simulink model "ADCS_FSM_v1_test"  (R2025b)
settings: Solver=VariableStepAuto  StartTime=0.0  StopTime=t0  FixedStep=0.1  MaxStep=0.1  RelTol=1e-3
model workspace (MAT data in the model file):
  i = 8
  omega_thr = 1
  simIn = Simulink.SimulationInput
  simIn.ExternalInput = Simulink.SimulationData.Dataset
  simIn.ExternalInput.any.Name = ''
  simIn.ExternalInput.any.Version = 3
  simIn.ExternalInput.any.Storage = Simulink.SimulationData.Storage.RamDatasetStorage
  simIn.ExternalInput.any.Storage.any.Version = 2
  simIn.ExternalInput.any.Storage.any.Elements{1} = timeseries
  simIn.ExternalInput.any.Storage.any.Elements{1}.Name = 'u1'
  simIn.ExternalInput.any.Storage.any.Elements{1}.DataInfo = tsdata.datametadata
  simIn.ExternalInput.any.Storage.any.Elements{1}.DataInfo.Interpolation = tsdata.interpolation
  simIn.ExternalInput.any.Storage.any.Elements{1}.DataInfo.Interpolation.Fhandle : function handle (value not decoded)
  simIn.ExternalInput.any.Storage.any.Elements{1}.DataInfo.Interpolation.Name = 'linear'
  simIn.ExternalInput.any.Storage.any.Elements{1}.TimeInfo = tsdata.timemetadata
  simIn.ExternalInput.any.Storage.any.Elements{1}.TimeInfo.Length = 101
  simIn.ExternalInput.any.Storage.any.Elements{1}.TimeInfo.DuplicateTimes = 0
  simIn.ExternalInput.any.Storage.any.Elements{1}.TimeInfo.Time_ = [0; 0.1; 0.2; 0.3; 0.4; 0.5; 0.6; 0.7; 0.8; 0.9; 1; 1.1; 1.2; 1.3; 1.4; 1.5; 1.6; 1.7; 1.8; 1.9; 2; 2.1; 2.2; 2.3; 2.4; 2.5; 2.6; 2.7; 2.8; 2.9; 3; 3.1; 3.2; 3.3; 3.4; 3.5; 3.6; 3.7; 3.8; 3.9; 4; 4.1; 4.2; 4.3; 4.4; 4.5; 4.6; 4.7; 4.8; 4.9; 5; 5.1; 5.2; 5.3; 5.4; 5.5; 5.6; 5.7; 5.8; 5.9; 6; 6.1; 6.2; 6.3; 6.4; 6.5; 6.6; 6.7; 6.8; 6.9; 7; 7.1; 7.2; 7.3; 7.4; 7.5; 7.6; 7.7; 7.8; 7.9; 8; 8.1; 8.2; 8.3; 8.4; 8.5; 8.6; 8.7; 8.8; 8.9; 9; 9.1; 9.2; 9.3; 9.4; 9.5; 9.6; 9.7; 9.8; 9.9; 10]
  simIn.ExternalInput.any.Storage.any.Elements{1}.TimeInfo.Initialized = 1
  simIn.ExternalInput.any.Storage.any.Elements{1}.QualityInfo = tsdata.qualmetadata
  simIn.ExternalInput.any.Storage.any.Elements{1}.Data_ = [12; 12; 12; 12; 12; 12; 12; 12; 12; 12; 12; 12; 12; 12; 12; 12; 12; 12; 12; 12; 12; 12; 12; 12; 12; 12; 12; 12; 12; 12; 12; 12; 12; 12; 12; 12; 12; 12; 12; 12; 12; 12; 12; 12; 12; 12; 12; 12; 12; 12; 12; 12; 12; 12; 12; 12; 12; 12; 12; 12; 12; 12; 12; 12; 12; 12; 12; 12; 12; 12; 12; 12; 12; 12; 12; 12; 12; 12; 12; 12; 12; 12; 12; 12; 12; 12; 12; 12; 12; 12; 12; 12; 12; 12; 12; 12; 12; 12; 12; 12; 12]
  simIn.ExternalInput.any.Storage.any.Elements{2} = timeseries
  simIn.ExternalInput.any.Storage.any.Elements{2}.Name = 'u2'
  simIn.ExternalInput.any.Storage.any.Elements{2}.DataInfo = tsdata.datametadata
  simIn.ExternalInput.any.Storage.any.Elements{2}.DataInfo.Interpolation = tsdata.interpolation
  simIn.ExternalInput.any.Storage.any.Elements{2}.DataInfo.Interpolation.Fhandle : function handle (value not decoded)
  simIn.ExternalInput.any.Storage.any.Elements{2}.DataInfo.Interpolation.Name = 'linear'
  simIn.ExternalInput.any.Storage.any.Elements{2}.TimeInfo = tsdata.timemetadata
  simIn.ExternalInput.any.Storage.any.Elements{2}.TimeInfo.Length = 101
  simIn.ExternalInput.any.Storage.any.Elements{2}.TimeInfo.DuplicateTimes = 0
  simIn.ExternalInput.any.Storage.any.Elements{2}.TimeInfo.Time_ = [0; 0.1; 0.2; 0.3; 0.4; 0.5; 0.6; 0.7; 0.8; 0.9; 1; 1.1; 1.2; 1.3; 1.4; 1.5; 1.6; 1.7; 1.8; 1.9; 2; 2.1; 2.2; 2.3; 2.4; 2.5; 2.6; 2.7; 2.8; 2.9; 3; 3.1; 3.2; 3.3; 3.4; 3.5; 3.6; 3.7; 3.8; 3.9; 4; 4.1; 4.2; 4.3; 4.4; 4.5; 4.6; 4.7; 4.8; 4.9; 5; 5.1; 5.2; 5.3; 5.4; 5.5; 5.6; 5.7; 5.8; 5.9; 6; 6.1; 6.2; 6.3; 6.4; 6.5; 6.6; 6.7; 6.8; 6.9; 7; 7.1; 7.2; 7.3; 7.4; 7.5; 7.6; 7.7; 7.8; 7.9; 8; 8.1; 8.2; 8.3; 8.4; 8.5; 8.6; 8.7; 8.8; 8.9; 9; 9.1; 9.2; 9.3; 9.4; 9.5; 9.6; 9.7; 9.8; 9.9; 10]
  simIn.ExternalInput.any.Storage.any.Elements{2}.TimeInfo.Initialized = 1
  simIn.ExternalInput.any.Storage.any.Elements{2}.QualityInfo = tsdata.qualmetadata
  simIn.ExternalInput.any.Storage.any.Elements{2}.Data_ = [1; 1; 1; 1; 1; 1; 1; 1; 1; 1; 1; 1; 1; 1; 1; 1; 1; 1; 1; 1; 1; 1; 1; 1; 1; 1; 1; 1; 1; 1; 1; 1; 1; 1; 1; 1; 1; 1; 1; 1; 1; 1; 1; 1; 1; 1; 1; 1; 1; 1; 1; 1; 1; 1; 1; 1; 1; 1; 1; 1; 1; 1; 1; 1; 1; 1; 1; 1; 1; 1; 1; 1; 1; 1; 1; 1; 1; 1; 1; 1; 1; 1; 1; 1; 1; 1; 1; 1; 1; 1; 1; 1; 1; 1; 1; 1; 1; 1; 1; 1; 1]
  simIn.ExternalInput.any.Storage.any.Elements{3} = timeseries
  simIn.ExternalInput.any.Storage.any.Elements{3}.Name = 'u3'
  simIn.ExternalInput.any.Storage.any.Elements{3}.DataInfo = tsdata.datametadata
  simIn.ExternalInput.any.Storage.any.Elements{3}.DataInfo.Interpolation = tsdata.interpolation
  simIn.ExternalInput.any.Storage.any.Elements{3}.DataInfo.Interpolation.Fhandle : function handle (value not decoded)
  simIn.ExternalInput.any.Storage.any.Elements{3}.DataInfo.Interpolation.Name = 'linear'
  simIn.ExternalInput.any.Storage.any.Elements{3}.TimeInfo = tsdata.timemetadata
  simIn.ExternalInput.any.Storage.any.Elements{3}.TimeInfo.Length = 101
  simIn.ExternalInput.any.Storage.any.Elements{3}.TimeInfo.DuplicateTimes = 0
  simIn.ExternalInput.any.Storage.any.Elements{3}.TimeInfo.Time_ = [0; 0.1; 0.2; 0.3; 0.4; 0.5; 0.6; 0.7; 0.8; 0.9; 1; 1.1; 1.2; 1.3; 1.4; 1.5; 1.6; 1.7; 1.8; 1.9; 2; 2.1; 2.2; 2.3; 2.4; 2.5; 2.6; 2.7; 2.8; 2.9; 3; 3.1; 3.2; 3.3; 3.4; 3.5; 3.6; 3.7; 3.8; 3.9; 4; 4.1; 4.2; 4.3; 4.4; 4.5; 4.6; 4.7; 4.8; 4.9; 5; 5.1; 5.2; 5.3; 5.4; 5.5; 5.6; 5.7; 5.8; 5.9; 6; 6.1; 6.2; 6.3; 6.4; 6.5; 6.6; 6.7; 6.8; 6.9; 7; 7.1; 7.2; 7.3; 7.4; 7.5; 7.6; 7.7; 7.8; 7.9; 8; 8.1; 8.2; 8.3; 8.4; 8.5; 8.6; 8.7; 8.8; 8.9; 9; 9.1; 9.2; 9.3; 9.4; 9.5; 9.6; 9.7; 9.8; 9.9; 10]
  simIn.ExternalInput.any.Storage.any.Elements{3}.TimeInfo.Initialized = 1
  simIn.ExternalInput.any.Storage.any.Elements{3}.QualityInfo = tsdata.qualmetadata
  simIn.ExternalInput.any.Storage.any.Elements{3}.Data_ = [0; 0; 0; 0; 0; 0; 0; 0; 0; 0; 0; 0; 0; 0; 0; 0; 0; 0; 0; 0; 0; 0; 0; 0; 0; 0; 0; 0; 0; 0; 0; 0; 0; 0; 0; 0; 0; 0; 0; 0; 0; 0; 0; 0; 0; 0; 0; 0; 0; 0; 0; 0; 0; 0; 0; 0; 0; 0; 0; 0; 0; 0; 0; 0; 0; 0; 0; 0; 0; 0; 0; 0; 0; 0; 0; 0; 0; 0; 0; 0; 0; 0; 0; 0; 0; 0; 0; 0; 0; 0; 0; 0; 0; 0; 0; 0; 0; 0; 0; 0; 0]
  simIn.ExternalInput.any.Storage.any.Elements{4} = timeseries
  simIn.ExternalInput.any.Storage.any.Elements{4}.Name = 'u4'
  simIn.ExternalInput.any.Storage.any.Elements{4}.DataInfo = tsdata.datametadata
  simIn.ExternalInput.any.Storage.any.Elements{4}.DataInfo.Interpolation = tsdata.interpolation
  simIn.ExternalInput.any.Storage.any.Elements{4}.DataInfo.Interpolation.Fhandle : function handle (value not decoded)
  simIn.ExternalInput.any.Storage.any.Elements{4}.DataInfo.Interpolation.Name = 'linear'
  simIn.ExternalInput.any.Storage.any.Elements{4}.TimeInfo = tsdata.timemetadata
  simIn.ExternalInput.any.Storage.any.Elements{4}.TimeInfo.Length = 101
  simIn.ExternalInput.any.Storage.any.Elements{4}.TimeInfo.DuplicateTimes = 0
  simIn.ExternalInput.any.Storage.any.Elements{4}.TimeInfo.Time_ = [0; 0.1; 0.2; 0.3; 0.4; 0.5; 0.6; 0.7; 0.8; 0.9; 1; 1.1; 1.2; 1.3; 1.4; 1.5; 1.6; 1.7; 1.8; 1.9; 2; 2.1; 2.2; 2.3; 2.4; 2.5; 2.6; 2.7; 2.8; 2.9; 3; 3.1; 3.2; 3.3; 3.4; 3.5; 3.6; 3.7; 3.8; 3.9; 4; 4.1; 4.2; 4.3; 4.4; 4.5; 4.6; 4.7; 4.8; 4.9; 5; 5.1; 5.2; 5.3; 5.4; 5.5; 5.6; 5.7; 5.8; 5.9; 6; 6.1; 6.2; 6.3; 6.4; 6.5; 6.6; 6.7; 6.8; 6.9; 7; 7.1; 7.2; 7.3; 7.4; 7.5; 7.6; 7.7; 7.8; 7.9; 8; 8.1; 8.2; 8.3; 8.4; 8.5; 8.6; 8.7; 8.8; 8.9; 9; 9.1; 9.2; 9.3; 9.4; 9.5; 9.6; 9.7; 9.8; 9.9; 10]
  simIn.ExternalInput.any.Storage.any.Elements{4}.TimeInfo.Initialized = 1
  simIn.ExternalInput.any.Storage.any.Elements{4}.QualityInfo = tsdata.qualmetadata
  simIn.ExternalInput.any.Storage.any.Elements{4}.Data_ = [1; 1; 1; 1; 1; 1; 1; 1; 1; 1; 1; 1; 1; 1; 1; 1; 1; 1; 1; 1; 1; 1; 1; 1; 1; 1; 1; 1; 1; 1; 1; 1; 1; 1; 1; 1; 1; 1; 1; 1; 1; 1; 1; 1; 1; 1; 1; 1; 1; 1; 1; 1; 1; 1; 1; 1; 1; 1; 1; 1; 1; 1; 1; 1; 1; 1; 1; 1; 1; 1; 1; 1; 1; 1; 1; 1; 1; 1; 1; 1; 1; 1; 1; 1; 1; 1; 1; 1; 1; 1; 1; 1; 1; 1; 1; 1; 1; 1; 1; 1; 1]
  simIn.ExternalInput.any.Storage.any.Elements{5} = timeseries
  simIn.ExternalInput.any.Storage.any.Elements{5}.Name = 'u5'
  simIn.ExternalInput.any.Storage.any.Elements{5}.DataInfo = tsdata.datametadata
  simIn.ExternalInput.any.Storage.any.Elements{5}.DataInfo.Interpolation = tsdata.interpolation
  simIn.ExternalInput.any.Storage.any.Elements{5}.DataInfo.Interpolation.Fhandle : function handle (value not decoded)
  simIn.ExternalInput.any.Storage.any.Elements{5}.DataInfo.Interpolation.Name = 'linear'
  simIn.ExternalInput.any.Storage.any.Elements{5}.TimeInfo = tsdata.timemetadata
  simIn.ExternalInput.any.Storage.any.Elements{5}.TimeInfo.Length = 101
  simIn.ExternalInput.any.Storage.any.Elements{5}.TimeInfo.DuplicateTimes = 0
  simIn.ExternalInput.any.Storage.any.Elements{5}.TimeInfo.Time_ = [0; 0.1; 0.2; 0.3; 0.4; 0.5; 0.6; 0.7; 0.8; 0.9; 1; 1.1; 1.2; 1.3; 1.4; 1.5; 1.6; 1.7; 1.8; 1.9; 2; 2.1; 2.2; 2.3; 2.4; 2.5; 2.6; 2.7; 2.8; 2.9; 3; 3.1; 3.2; 3.3; 3.4; 3.5; 3.6; 3.7; 3.8; 3.9; 4; 4.1; 4.2; 4.3; 4.4; 4.5; 4.6; 4.7; 4.8; 4.9; 5; 5.1; 5.2; 5.3; 5.4; 5.5; 5.6; 5.7; 5.8; 5.9; 6; 6.1; 6.2; 6.3; 6.4; 6.5; 6.6; 6.7; 6.8; 6.9; 7; 7.1; 7.2; 7.3; 7.4; 7.5; 7.6; 7.7; 7.8; 7.9; 8; 8.1; 8.2; 8.3; 8.4; 8.5; 8.6; 8.7; 8.8; 8.9; 9; 9.1; 9.2; 9.3; 9.4; 9.5; 9.6; 9.7; 9.8; 9.9; 10]
  simIn.ExternalInput.any.Storage.any.Elements{5}.TimeInfo.Initialized = 1
  simIn.ExternalInput.any.Storage.any.Elements{5}.QualityInfo = tsdata.qualmetadata
  simIn.ExternalInput.any.Storage.any.Elements{5}.Data_ = [0; 0; 0; 0; 0; 0; 0; 0; 0; 0; 0; 0; 0; 0; 0; 0; 0; 0; 0; 0; 0; 0; 0; 0; 0; 0; 0; 0; 0; 0; 0; 0; 0; 0; 0; 0; 0; 0; 0; 0; 0; 0; 0; 0; 0; 0; 0; 0; 0; 0; 0; 0; 0; 0; 0; 0; 0; 0; 0; 0; 0; 0; 0; 0; 0; 0; 0; 0; 0; 0; 0; 0; 0; 0; 0; 0; 0; 0; 0; 0; 0; 0; 0; 0; 0; 0; 0; 0; 0; 0; 0; 0; 0; 0; 0; 0; 0; 0; 0; 0; 0]
  simIn.ExternalInput.any.Storage.any.Elements{6} = timeseries
  simIn.ExternalInput.any.Storage.any.Elements{6}.Name = 'u6'
  simIn.ExternalInput.any.Storage.any.Elements{6}.DataInfo = tsdata.datametadata
  simIn.ExternalInput.any.Storage.any.Elements{6}.DataInfo.Interpolation = tsdata.interpolation
  simIn.ExternalInput.any.Storage.any.Elements{6}.DataInfo.Interpolation.Fhandle : function handle (value not decoded)
  simIn.ExternalInput.any.Storage.any.Elements{6}.DataInfo.Interpolation.Name = 'linear'
  simIn.ExternalInput.any.Storage.any.Elements{6}.TimeInfo = tsdata.timemetadata
  simIn.ExternalInput.any.Storage.any.Elements{6}.TimeInfo.Length = 101
  simIn.ExternalInput.any.Storage.any.Elements{6}.TimeInfo.DuplicateTimes = 0
  simIn.ExternalInput.any.Storage.any.Elements{6}.TimeInfo.Time_ = [0; 0.1; 0.2; 0.3; 0.4; 0.5; 0.6; 0.7; 0.8; 0.9; 1; 1.1; 1.2; 1.3; 1.4; 1.5; 1.6; 1.7; 1.8; 1.9; 2; 2.1; 2.2; 2.3; 2.4; 2.5; 2.6; 2.7; 2.8; 2.9; 3; 3.1; 3.2; 3.3; 3.4; 3.5; 3.6; 3.7; 3.8; 3.9; 4; 4.1; 4.2; 4.3; 4.4; 4.5; 4.6; 4.7; 4.8; 4.9; 5; 5.1; 5.2; 5.3; 5.4; 5.5; 5.6; 5.7; 5.8; 5.9; 6; 6.1; 6.2; 6.3; 6.4; 6.5; 6.6; 6.7; 6.8; 6.9; 7; 7.1; 7.2; 7.3; 7.4; 7.5; 7.6; 7.7; 7.8; 7.9; 8; 8.1; 8.2; 8.3; 8.4; 8.5; 8.6; 8.7; 8.8; 8.9; 9; 9.1; 9.2; 9.3; 9.4; 9.5; 9.6; 9.7; 9.8; 9.9; 10]
  simIn.ExternalInput.any.Storage.any.Elements{6}.TimeInfo.Initialized = 1
  simIn.ExternalInput.any.Storage.any.Elements{6}.QualityInfo = tsdata.qualmetadata
  simIn.ExternalInput.any.Storage.any.Elements{6}.Data_ = [1; 1; 1; 1; 1; 1; 1; 1; 1; 1; 1; 1; 1; 1; 1; 1; 1; 1; 1; 1; 1; 1; 1; 1; 1; 1; 1; 1; 1; 1; 1; 1; 1; 1; 1; 1; 1; 1; 1; 1; 1; 1; 1; 1; 1; 1; 1; 1; 1; 1; 1; 1; 1; 1; 1; 1; 1; 1; 1; 1; 1; 1; 1; 1; 1; 1; 1; 1; 1; 1; 1; 1; 1; 1; 1; 1; 1; 1; 1; 1; 1; 1; 1; 1; 1; 1; 1; 1; 1; 1; 1; 1; 1; 1; 1; 1; 1; 1; 1; 1; 1]
  simIn.ExternalInput.any.Storage.any.Elements{7} = timeseries
  simIn.ExternalInput.any.Storage.any.Elements{7}.Name = 'u7'
  simIn.ExternalInput.any.Storage.any.Elements{7}.DataInfo = tsdata.datametadata
  simIn.ExternalInput.any.Storage.any.Elements{7}.DataInfo.Interpolation = tsdata.interpolation
  simIn.ExternalInput.any.Storage.any.Elements{7}.DataInfo.Interpolation.Fhandle : function handle (value not decoded)
  simIn.ExternalInput.any.Storage.any.Elements{7}.DataInfo.Interpolation.Name = 'linear'
  simIn.ExternalInput.any.Storage.any.Elements{7}.TimeInfo = tsdata.timemetadata
  simIn.ExternalInput.any.Storage.any.Elements{7}.TimeInfo.Length = 101
  simIn.ExternalInput.any.Storage.any.Elements{7}.TimeInfo.DuplicateTimes = 0
  simIn.ExternalInput.any.Storage.any.Elements{7}.TimeInfo.Time_ = [0; 0.1; 0.2; 0.3; 0.4; 0.5; 0.6; 0.7; 0.8; 0.9; 1; 1.1; 1.2; 1.3; 1.4; 1.5; 1.6; 1.7; 1.8; 1.9; 2; 2.1; 2.2; 2.3; 2.4; 2.5; 2.6; 2.7; 2.8; 2.9; 3; 3.1; 3.2; 3.3; 3.4; 3.5; 3.6; 3.7; 3.8; 3.9; 4; 4.1; 4.2; 4.3; 4.4; 4.5; 4.6; 4.7; 4.8; 4.9; 5; 5.1; 5.2; 5.3; 5.4; 5.5; 5.6; 5.7; 5.8; 5.9; 6; 6.1; 6.2; 6.3; 6.4; 6.5; 6.6; 6.7; 6.8; 6.9; 7; 7.1; 7.2; 7.3; 7.4; 7.5; 7.6; 7.7; 7.8; 7.9; 8; 8.1; 8.2; 8.3; 8.4; 8.5; 8.6; 8.7; 8.8; 8.9; 9; 9.1; 9.2; 9.3; 9.4; 9.5; 9.6; 9.7; 9.8; 9.9; 10]
  simIn.ExternalInput.any.Storage.any.Elements{7}.TimeInfo.Initialized = 1
  simIn.ExternalInput.any.Storage.any.Elements{7}.QualityInfo = tsdata.qualmetadata
  simIn.ExternalInput.any.Storage.any.Elements{7}.Data_ = [1; 1; 1; 1; 1; 1; 1; 1; 1; 1; 1; 1; 1; 1; 1; 1; 1; 1; 1; 1; 1; 1; 1; 1; 1; 1; 1; 1; 1; 1; 1; 1; 1; 1; 1; 1; 1; 1; 1; 1; 1; 1; 1; 1; 1; 1; 1; 1; 1; 1; 1; 1; 1; 1; 1; 1; 1; 1; 1; 1; 1; 1; 1; 1; 1; 1; 1; 1; 1; 1; 1; 1; 1; 1; 1; 1; 1; 1; 1; 1; 1; 1; 1; 1; 1; 1; 1; 1; 1; 1; 1; 1; 1; 1; 1; 1; 1; 1; 1; 1; 1]
  simIn.ExternalInput.any.Storage.any.Elements{8} = timeseries
  simIn.ExternalInput.any.Storage.any.Elements{8}.Name = 'u8'
  simIn.ExternalInput.any.Storage.any.Elements{8}.DataInfo = tsdata.datametadata
  simIn.ExternalInput.any.Storage.any.Elements{8}.DataInfo.Interpolation = tsdata.interpolation
  simIn.ExternalInput.any.Storage.any.Elements{8}.DataInfo.Interpolation.Fhandle : function handle (value not decoded)
  simIn.ExternalInput.any.Storage.any.Elements{8}.DataInfo.Interpolation.Name = 'linear'
  simIn.ExternalInput.any.Storage.any.Elements{8}.TimeInfo = tsdata.timemetadata
  simIn.ExternalInput.any.Storage.any.Elements{8}.TimeInfo.Length = 101
  simIn.ExternalInput.any.Storage.any.Elements{8}.TimeInfo.DuplicateTimes = 0
  simIn.ExternalInput.any.Storage.any.Elements{8}.TimeInfo.Time_ = [0; 0.1; 0.2; 0.3; 0.4; 0.5; 0.6; 0.7; 0.8; 0.9; 1; 1.1; 1.2; 1.3; 1.4; 1.5; 1.6; 1.7; 1.8; 1.9; 2; 2.1; 2.2; 2.3; 2.4; 2.5; 2.6; 2.7; 2.8; 2.9; 3; 3.1; 3.2; 3.3; 3.4; 3.5; 3.6; 3.7; 3.8; 3.9; 4; 4.1; 4.2; 4.3; 4.4; 4.5; 4.6; 4.7; 4.8; 4.9; 5; 5.1; 5.2; 5.3; 5.4; 5.5; 5.6; 5.7; 5.8; 5.9; 6; 6.1; 6.2; 6.3; 6.4; 6.5; 6.6; 6.7; 6.8; 6.9; 7; 7.1; 7.2; 7.3; 7.4; 7.5; 7.6; 7.7; 7.8; 7.9; 8; 8.1; 8.2; 8.3; 8.4; 8.5; 8.6; 8.7; 8.8; 8.9; 9; 9.1; 9.2; 9.3; 9.4; 9.5; 9.6; 9.7; 9.8; 9.9; 10]
  simIn.ExternalInput.any.Storage.any.Elements{8}.TimeInfo.Initialized = 1
  simIn.ExternalInput.any.Storage.any.Elements{8}.QualityInfo = tsdata.qualmetadata
  simIn.ExternalInput.any.Storage.any.Elements{8}.Data_ = [0; 0; 0; 0; 0; 0; 0; 0; 0; 0; 0; 0; 0; 0; 0; 0; 0; 0; 0; 0; 0; 0; 0; 0; 0; 0; 0; 0; 0; 0; 0; 0; 0; 0; 0; 0; 0; 0; 0; 0; 0; 0; 0; 0; 0; 0; 0; 0; 0; 0; 0; 0; 0; 0; 0; 0; 0; 0; 0; 0; 0; 0; 0; 0; 0; 0; 0; 0; 0; 0; 0; 0; 0; 0; 0; 0; 0; 0; 0; 0; 0; 0; 0; 0; 0; 0; 0; 0; 0; 0; 0; 0; 0; 0; 0; 0; 0; 0; 0; 0; 0]
  simIn.ExternalInput.any.Storage.any.Elements{9} = timeseries
  simIn.ExternalInput.any.Storage.any.Elements{9}.Name = 'u9'
  simIn.ExternalInput.any.Storage.any.Elements{9}.DataInfo = tsdata.datametadata
  simIn.ExternalInput.any.Storage.any.Elements{9}.DataInfo.Interpolation = tsdata.interpolation
  simIn.ExternalInput.any.Storage.any.Elements{9}.DataInfo.Interpolation.Fhandle : function handle (value not decoded)
  simIn.ExternalInput.any.Storage.any.Elements{9}.DataInfo.Interpolation.Name = 'linear'
  simIn.ExternalInput.any.Storage.any.Elements{9}.TimeInfo = tsdata.timemetadata
  simIn.ExternalInput.any.Storage.any.Elements{9}.TimeInfo.Length = 101
  simIn.ExternalInput.any.Storage.any.Elements{9}.TimeInfo.DuplicateTimes = 0
  simIn.ExternalInput.any.Storage.any.Elements{9}.TimeInfo.Time_ = [0; 0.1; 0.2; 0.3; 0.4; 0.5; 0.6; 0.7; 0.8; 0.9; 1; 1.1; 1.2; 1.3; 1.4; 1.5; 1.6; 1.7; 1.8; 1.9; 2; 2.1; 2.2; 2.3; 2.4; 2.5; 2.6; 2.7; 2.8; 2.9; 3; 3.1; 3.2; 3.3; 3.4; 3.5; 3.6; 3.7; 3.8; 3.9; 4; 4.1; 4.2; 4.3; 4.4; 4.5; 4.6; 4.7; 4.8; 4.9; 5; 5.1; 5.2; 5.3; 5.4; 5.5; 5.6; 5.7; 5.8; 5.9; 6; 6.1; 6.2; 6.3; 6.4; 6.5; 6.6; 6.7; 6.8; 6.9; 7; 7.1; 7.2; 7.3; 7.4; 7.5; 7.6; 7.7; 7.8; 7.9; 8; 8.1; 8.2; 8.3; 8.4; 8.5; 8.6; 8.7; 8.8; 8.9; 9; 9.1; 9.2; 9.3; 9.4; 9.5; 9.6; 9.7; 9.8; 9.9; 10]
  simIn.ExternalInput.any.Storage.any.Elements{9}.TimeInfo.Initialized = 1
  simIn.ExternalInput.any.Storage.any.Elements{9}.QualityInfo = tsdata.qualmetadata
  simIn.ExternalInput.any.Storage.any.Elements{9}.Data_ = [1; 1; 1; 1; 1; 1; 1; 1; 1; 1; 1; 1; 1; 1; 1; 1; 1; 1; 1; 1; 1; 1; 1; 1; 1; 1; 1; 1; 1; 1; 1; 1; 1; 1; 1; 1; 1; 1; 1; 1; 1; 1; 1; 1; 1; 1; 1; 1; 1; 1; 1; 1; 1; 1; 1; 1; 1; 1; 1; 1; 1; 1; 1; 1; 1; 1; 1; 1; 1; 1; 1; 1; 1; 1; 1; 1; 1; 1; 1; 1; 1; 1; 1; 1; 1; 1; 1; 1; 1; 1; 1; 1; 1; 1; 1; 1; 1; 1; 1; 1; 1]
  simIn.ExternalInput.any.Storage.any.Elements{10} = timeseries
  simIn.ExternalInput.any.Storage.any.Elements{10}.Name = 'u10'
  simIn.ExternalInput.any.Storage.any.Elements{10}.DataInfo = tsdata.datametadata
  simIn.ExternalInput.any.Storage.any.Elements{10}.DataInfo.Interpolation = tsdata.interpolation
  simIn.ExternalInput.any.Storage.any.Elements{10}.DataInfo.Interpolation.Fhandle : function handle (value not decoded)
  simIn.ExternalInput.any.Storage.any.Elements{10}.DataInfo.Interpolation.Name = 'linear'
  simIn.ExternalInput.any.Storage.any.Elements{10}.TimeInfo = tsdata.timemetadata
  simIn.ExternalInput.any.Storage.any.Elements{10}.TimeInfo.Length = 101
  simIn.ExternalInput.any.Storage.any.Elements{10}.TimeInfo.DuplicateTimes = 0
  simIn.ExternalInput.any.Storage.any.Elements{10}.TimeInfo.Time_ = [0; 0.1; 0.2; 0.3; 0.4; 0.5; 0.6; 0.7; 0.8; 0.9; 1; 1.1; 1.2; 1.3; 1.4; 1.5; 1.6; 1.7; 1.8; 1.9; 2; 2.1; 2.2; 2.3; 2.4; 2.5; 2.6; 2.7; 2.8; 2.9; 3; 3.1; 3.2; 3.3; 3.4; 3.5; 3.6; 3.7; 3.8; 3.9; 4; 4.1; 4.2; 4.3; 4.4; 4.5; 4.6; 4.7; 4.8; 4.9; 5; 5.1; 5.2; 5.3; 5.4; 5.5; 5.6; 5.7; 5.8; 5.9; 6; 6.1; 6.2; 6.3; 6.4; 6.5; 6.6; 6.7; 6.8; 6.9; 7; 7.1; 7.2; 7.3; 7.4; 7.5; 7.6; 7.7; 7.8; 7.9; 8; 8.1; 8.2; 8.3; 8.4; 8.5; 8.6; 8.7; 8.8; 8.9; 9; 9.1; 9.2; 9.3; 9.4; 9.5; 9.6; 9.7; 9.8; 9.9; 10]
  simIn.ExternalInput.any.Storage.any.Elements{10}.TimeInfo.Initialized = 1
  simIn.ExternalInput.any.Storage.any.Elements{10}.QualityInfo = tsdata.qualmetadata
  simIn.ExternalInput.any.Storage.any.Elements{10}.Data_ = [0; 0; 0; 0; 0; 0; 0; 0; 0; 0; 0; 0; 0; 0; 0; 0; 0; 0; 0; 0; 0; 0; 0; 0; 0; 0; 0; 0; 0; 0; 0; 0; 0; 0; 0; 0; 0; 0; 0; 0; 0; 0; 0; 0; 0; 0; 0; 0; 0; 0; 0; 0; 0; 0; 0; 0; 0; 0; 0; 0; 0; 0; 0; 0; 0; 0; 0; 0; 0; 0; 0; 0; 0; 0; 0; 0; 0; 0; 0; 0; 0; 0; 0; 0; 0; 0; 0; 0; 0; 0; 0; 0; 0; 0; 0; 0; 0; 0; 0; 0; 0]
  simIn.ExternalInput.any.Storage.any.Elements{11} = timeseries
  simIn.ExternalInput.any.Storage.any.Elements{11}.Name = 'u11'
  simIn.ExternalInput.any.Storage.any.Elements{11}.DataInfo = tsdata.datametadata
  simIn.ExternalInput.any.Storage.any.Elements{11}.DataInfo.Interpolation = tsdata.interpolation
  simIn.ExternalInput.any.Storage.any.Elements{11}.DataInfo.Interpolation.Fhandle : function handle (value not decoded)
  simIn.ExternalInput.any.Storage.any.Elements{11}.DataInfo.Interpolation.Name = 'linear'
  simIn.ExternalInput.any.Storage.any.Elements{11}.TimeInfo = tsdata.timemetadata
  simIn.ExternalInput.any.Storage.any.Elements{11}.TimeInfo.Length = 101
  simIn.ExternalInput.any.Storage.any.Elements{11}.TimeInfo.DuplicateTimes = 0
  simIn.ExternalInput.any.Storage.any.Elements{11}.TimeInfo.Time_ = [0; 0.1; 0.2; 0.3; 0.4; 0.5; 0.6; 0.7; 0.8; 0.9; 1; 1.1; 1.2; 1.3; 1.4; 1.5; 1.6; 1.7; 1.8; 1.9; 2; 2.1; 2.2; 2.3; 2.4; 2.5; 2.6; 2.7; 2.8; 2.9; 3; 3.1; 3.2; 3.3; 3.4; 3.5; 3.6; 3.7; 3.8; 3.9; 4; 4.1; 4.2; 4.3; 4.4; 4.5; 4.6; 4.7; 4.8; 4.9; 5; 5.1; 5.2; 5.3; 5.4; 5.5; 5.6; 5.7; 5.8; 5.9; 6; 6.1; 6.2; 6.3; 6.4; 6.5; 6.6; 6.7; 6.8; 6.9; 7; 7.1; 7.2; 7.3; 7.4; 7.5; 7.6; 7.7; 7.8; 7.9; 8; 8.1; 8.2; 8.3; 8.4; 8.5; 8.6; 8.7; 8.8; 8.9; 9; 9.1; 9.2; 9.3; 9.4; 9.5; 9.6; 9.7; 9.8; 9.9; 10]
  simIn.ExternalInput.any.Storage.any.Elements{11}.TimeInfo.Initialized = 1
  simIn.ExternalInput.any.Storage.any.Elements{11}.QualityInfo = tsdata.qualmetadata
  simIn.ExternalInput.any.Storage.any.Elements{11}.Data_ = [1; 1; 1; 1; 1; 1; 1; 1; 1; 1; 1; 1; 1; 1; 1; 1; 1; 1; 1; 1; 1; 1; 1; 1; 1; 1; 1; 1; 1; 1; 1; 1; 1; 1; 1; 1; 1; 1; 1; 1; 1; 1; 1; 1; 1; 1; 1; 1; 1; 1; 1; 1; 1; 1; 1; 1; 1; 1; 1; 1; 1; 1; 1; 1; 1; 1; 1; 1; 1; 1; 1; 1; 1; 1; 1; 1; 1; 1; 1; 1; 1; 1; 1; 1; 1; 1; 1; 1; 1; 1; 1; 1; 1; 1; 1; 1; 1; 1; 1; 1; 1]
  simIn.ExternalInput.any.Storage.any.Elements{12} = timeseries
  simIn.ExternalInput.any.Storage.any.Elements{12}.Name = 'u12'
  simIn.ExternalInput.any.Storage.any.Elements{12}.DataInfo = tsdata.datametadata
  simIn.ExternalInput.any.Storage.any.Elements{12}.DataInfo.Interpolation = tsdata.interpolation
  simIn.ExternalInput.any.Storage.any.Elements{12}.DataInfo.Interpolation.Fhandle : function handle (value not decoded)
  simIn.ExternalInput.any.Storage.any.Elements{12}.DataInfo.Interpolation.Name = 'linear'
  simIn.ExternalInput.any.Storage.any.Elements{12}.TimeInfo = tsdata.timemetadata
  simIn.ExternalInput.any.Storage.any.Elements{12}.TimeInfo.Length = 101
  simIn.ExternalInput.any.Storage.any.Elements{12}.TimeInfo.DuplicateTimes = 0
  simIn.ExternalInput.any.Storage.any.Elements{12}.TimeInfo.Time_ = [0; 0.1; 0.2; 0.3; 0.4; 0.5; 0.6; 0.7; 0.8; 0.9; 1; 1.1; 1.2; 1.3; 1.4; 1.5; 1.6; 1.7; 1.8; 1.9; 2; 2.1; 2.2; 2.3; 2.4; 2.5; 2.6; 2.7; 2.8; 2.9; 3; 3.1; 3.2; 3.3; 3.4; 3.5; 3.6; 3.7; 3.8; 3.9; 4; 4.1; 4.2; 4.3; 4.4; 4.5; 4.6; 4.7; 4.8; 4.9; 5; 5.1; 5.2; 5.3; 5.4; 5.5; 5.6; 5.7; 5.8; 5.9; 6; 6.1; 6.2; 6.3; 6.4; 6.5; 6.6; 6.7; 6.8; 6.9; 7; 7.1; 7.2; 7.3; 7.4; 7.5; 7.6; 7.7; 7.8; 7.9; 8; 8.1; 8.2; 8.3; 8.4; 8.5; 8.6; 8.7; 8.8; 8.9; 9; 9.1; 9.2; 9.3; 9.4; 9.5; 9.6; 9.7; 9.8; 9.9; 10]
  simIn.ExternalInput.any.Storage.any.Elements{12}.TimeInfo.Initialized = 1
  simIn.ExternalInput.any.Storage.any.Elements{12}.QualityInfo = tsdata.qualmetadata
  simIn.ExternalInput.any.Storage.any.Elements{12}.Data_ = [1; 1; 1; 1; 1; 1; 1; 1; 1; 1; 1; 1; 1; 1; 1; 1; 1; 1; 1; 1; 1; 1; 1; 1; 1; 1; 1; 1; 1; 1; 1; 1; 1; 1; 1; 1; 1; 1; 1; 1; 1; 1; 1; 1; 1; 1; 1; 1; 1; 1; 1; 1; 1; 1; 1; 1; 1; 1; 1; 1; 1; 1; 1; 1; 1; 1; 1; 1; 1; 1; 1; 1; 1; 1; 1; 1; 1; 1; 1; 1; 1; 1; 1; 1; 1; 1; 1; 1; 1; 1; 1; 1; 1; 1; 1; 1; 1; 1; 1; 1; 1]
  simIn.ExternalInput.any.Storage.any.Elements{13} = timeseries
  simIn.ExternalInput.any.Storage.any.Elements{13}.Name = 'u13'
  simIn.ExternalInput.any.Storage.any.Elements{13}.DataInfo = tsdata.datametadata
  simIn.ExternalInput.any.Storage.any.Elements{13}.DataInfo.Interpolation = tsdata.interpolation
  simIn.ExternalInput.any.Storage.any.Elements{13}.DataInfo.Interpolation.Fhandle : function handle (value not decoded)
  simIn.ExternalInput.any.Storage.any.Elements{13}.DataInfo.Interpolation.Name = 'linear'
  simIn.ExternalInput.any.Storage.any.Elements{13}.TimeInfo = tsdata.timemetadata
  simIn.ExternalInput.any.Storage.any.Elements{13}.TimeInfo.Length = 101
  simIn.ExternalInput.any.Storage.any.Elements{13}.TimeInfo.DuplicateTimes = 0
  simIn.ExternalInput.any.Storage.any.Elements{13}.TimeInfo.Time_ = [0; 0.1; 0.2; 0.3; 0.4; 0.5; 0.6; 0.7; 0.8; 0.9; 1; 1.1; 1.2; 1.3; 1.4; 1.5; 1.6; 1.7; 1.8; 1.9; 2; 2.1; 2.2; 2.3; 2.4; 2.5; 2.6; 2.7; 2.8; 2.9; 3; 3.1; 3.2; 3.3; 3.4; 3.5; 3.6; 3.7; 3.8; 3.9; 4; 4.1; 4.2; 4.3; 4.4; 4.5; 4.6; 4.7; 4.8; 4.9; 5; 5.1; 5.2; 5.3; 5.4; 5.5; 5.6; 5.7; 5.8; 5.9; 6; 6.1; 6.2; 6.3; 6.4; 6.5; 6.6; 6.7; 6.8; 6.9; 7; 7.1; 7.2; 7.3; 7.4; 7.5; 7.6; 7.7; 7.8; 7.9; 8; 8.1; 8.2; 8.3; 8.4; 8.5; 8.6; 8.7; 8.8; 8.9; 9; 9.1; 9.2; 9.3; 9.4; 9.5; 9.6; 9.7; 9.8; 9.9; 10]
  simIn.ExternalInput.any.Storage.any.Elements{13}.TimeInfo.Initialized = 1
  simIn.ExternalInput.any.Storage.any.Elements{13}.QualityInfo = tsdata.qualmetadata
  simIn.ExternalInput.any.Storage.any.Elements{13}.Data_ = [1; 1; 1; 1; 1; 1; 1; 1; 1; 1; 1; 1; 1; 1; 1; 1; 1; 1; 1; 1; 1; 1; 1; 1; 1; 1; 1; 1; 1; 1; 1; 1; 1; 1; 1; 1; 1; 1; 1; 1; 1; 1; 1; 1; 1; 1; 1; 1; 1; 1; 1; 1; 1; 1; 1; 1; 1; 1; 1; 1; 1; 1; 1; 1; 1; 1; 1; 1; 1; 1; 1; 1; 1; 1; 1; 1; 1; 1; 1; 1; 1; 1; 1; 1; 1; 1; 1; 1; 1; 1; 1; 1; 1; 1; 1; 1; 1; 1; 1; 1; 1]
  simIn.ExternalInput.any.Storage.any.Elements{14} = timeseries
  simIn.ExternalInput.any.Storage.any.Elements{14}.Name = 'u14'
  simIn.ExternalInput.any.Storage.any.Elements{14}.DataInfo = tsdata.datametadata
  simIn.ExternalInput.any.Storage.any.Elements{14}.DataInfo.Interpolation = tsdata.interpolation
  simIn.ExternalInput.any.Storage.any.Elements{14}.DataInfo.Interpolation.Fhandle : function handle (value not decoded)
  simIn.ExternalInput.any.Storage.any.Elements{14}.DataInfo.Interpolation.Name = 'linear'
  simIn.ExternalInput.any.Storage.any.Elements{14}.TimeInfo = tsdata.timemetadata
  simIn.ExternalInput.any.Storage.any.Elements{14}.TimeInfo.Length = 101
  simIn.ExternalInput.any.Storage.any.Elements{14}.TimeInfo.DuplicateTimes = 0
  simIn.ExternalInput.any.Storage.any.Elements{14}.TimeInfo.Time_ = [0; 0.1; 0.2; 0.3; 0.4; 0.5; 0.6; 0.7; 0.8; 0.9; 1; 1.1; 1.2; 1.3; 1.4; 1.5; 1.6; 1.7; 1.8; 1.9; 2; 2.1; 2.2; 2.3; 2.4; 2.5; 2.6; 2.7; 2.8; 2.9; 3; 3.1; 3.2; 3.3; 3.4; 3.5; 3.6; 3.7; 3.8; 3.9; 4; 4.1; 4.2; 4.3; 4.4; 4.5; 4.6; 4.7; 4.8; 4.9; 5; 5.1; 5.2; 5.3; 5.4; 5.5; 5.6; 5.7; 5.8; 5.9; 6; 6.1; 6.2; 6.3; 6.4; 6.5; 6.6; 6.7; 6.8; 6.9; 7; 7.1; 7.2; 7.3; 7.4; 7.5; 7.6; 7.7; 7.8; 7.9; 8; 8.1; 8.2; 8.3; 8.4; 8.5; 8.6; 8.7; 8.8; 8.9; 9; 9.1; 9.2; 9.3; 9.4; 9.5; 9.6; 9.7; 9.8; 9.9; 10]
  simIn.ExternalInput.any.Storage.any.Elements{14}.TimeInfo.Initialized = 1
  simIn.ExternalInput.any.Storage.any.Elements{14}.QualityInfo = tsdata.qualmetadata
  simIn.ExternalInput.any.Storage.any.Elements{14}.Data_ = [1; 1; 1; 1; 1; 1; 1; 1; 1; 1; 1; 1; 1; 1; 1; 1; 1; 1; 1; 1; 1; 1; 1; 1; 1; 1; 1; 1; 1; 1; 1; 1; 1; 1; 1; 1; 1; 1; 1; 1; 1; 1; 1; 1; 1; 1; 1; 1; 1; 1; 1; 1; 1; 1; 1; 1; 1; 1; 1; 1; 1; 1; 1; 1; 1; 1; 1; 1; 1; 1; 1; 1; 1; 1; 1; 1; 1; 1; 1; 1; 1; 1; 1; 1; 1; 1; 1; 1; 1; 1; 1; 1; 1; 1; 1; 1; 1; 1; 1; 1; 1]
  simIn.ExternalInput.any.Storage.any.Elements{15} = timeseries
  simIn.ExternalInput.any.Storage.any.Elements{15}.Name = 'u15'
  simIn.ExternalInput.any.Storage.any.Elements{15}.DataInfo = tsdata.datametadata
  simIn.ExternalInput.any.Storage.any.Elements{15}.DataInfo.Interpolation = tsdata.interpolation
  simIn.ExternalInput.any.Storage.any.Elements{15}.DataInfo.Interpolation.Fhandle : function handle (value not decoded)
  simIn.ExternalInput.any.Storage.any.Elements{15}.DataInfo.Interpolation.Name = 'linear'
  simIn.ExternalInput.any.Storage.any.Elements{15}.TimeInfo = tsdata.timemetadata
  simIn.ExternalInput.any.Storage.any.Elements{15}.TimeInfo.Length = 101
  simIn.ExternalInput.any.Storage.any.Elements{15}.TimeInfo.DuplicateTimes = 0
  simIn.ExternalInput.any.Storage.any.Elements{15}.TimeInfo.Time_ = [0; 0.1; 0.2; 0.3; 0.4; 0.5; 0.6; 0.7; 0.8; 0.9; 1; 1.1; 1.2; 1.3; 1.4; 1.5; 1.6; 1.7; 1.8; 1.9; 2; 2.1; 2.2; 2.3; 2.4; 2.5; 2.6; 2.7; 2.8; 2.9; 3; 3.1; 3.2; 3.3; 3.4; 3.5; 3.6; 3.7; 3.8; 3.9; 4; 4.1; 4.2; 4.3; 4.4; 4.5; 4.6; 4.7; 4.8; 4.9; 5; 5.1; 5.2; 5.3; 5.4; 5.5; 5.6; 5.7; 5.8; 5.9; 6; 6.1; 6.2; 6.3; 6.4; 6.5; 6.6; 6.7; 6.8; 6.9; 7; 7.1; 7.2; 7.3; 7.4; 7.5; 7.6; 7.7; 7.8; 7.9; 8; 8.1; 8.2; 8.3; 8.4; 8.5; 8.6; 8.7; 8.8; 8.9; 9; 9.1; 9.2; 9.3; 9.4; 9.5; 9.6; 9.7; 9.8; 9.9; 10]
  simIn.ExternalInput.any.Storage.any.Elements{15}.TimeInfo.Initialized = 1
  simIn.ExternalInput.any.Storage.any.Elements{15}.QualityInfo = tsdata.qualmetadata
  simIn.ExternalInput.any.Storage.any.Elements{15}.Data_ = [1; 1; 1; 1; 1; 1; 1; 1; 1; 1; 1; 1; 1; 1; 1; 1; 1; 1; 1; 1; 1; 1; 1; 1; 1; 1; 1; 1; 1; 1; 1; 1; 1; 1; 1; 1; 1; 1; 1; 1; 1; 1; 1; 1; 1; 1; 1; 1; 1; 1; 1; 1; 1; 1; 1; 1; 1; 1; 1; 1; 1; 1; 1; 1; 1; 1; 1; 1; 1; 1; 1; 1; 1; 1; 1; 1; 1; 1; 1; 1; 1; 1; 1; 1; 1; 1; 1; 1; 1; 1; 1; 1; 1; 1; 1; 1; 1; 1; 1; 1; 1]
  simIn.ExternalInput.any.Storage.any.Elements{16} = timeseries
  simIn.ExternalInput.any.Storage.any.Elements{16}.Name = 'u16'
  simIn.ExternalInput.any.Storage.any.Elements{16}.DataInfo = tsdata.datametadata
  simIn.ExternalInput.any.Storage.any.Elements{16}.DataInfo.Interpolation = tsdata.interpolation
  simIn.ExternalInput.any.Storage.any.Elements{16}.DataInfo.Interpolation.Fhandle : function handle (value not decoded)
  simIn.ExternalInput.any.Storage.any.Elements{16}.DataInfo.Interpolation.Name = 'linear'
  simIn.ExternalInput.any.Storage.any.Elements{16}.TimeInfo = tsdata.timemetadata
  simIn.ExternalInput.any.Storage.any.Elements{16}.TimeInfo.Length = 101
  simIn.ExternalInput.any.Storage.any.Elements{16}.TimeInfo.DuplicateTimes = 0
  simIn.ExternalInput.any.Storage.any.Elements{16}.TimeInfo.Time_ = [0; 0.1; 0.2; 0.3; 0.4; 0.5; 0.6; 0.7; 0.8; 0.9; 1; 1.1; 1.2; 1.3; 1.4; 1.5; 1.6; 1.7; 1.8; 1.9; 2; 2.1; 2.2; 2.3; 2.4; 2.5; 2.6; 2.7; 2.8; 2.9; 3; 3.1; 3.2; 3.3; 3.4; 3.5; 3.6; 3.7; 3.8; 3.9; 4; 4.1; 4.2; 4.3; 4.4; 4.5; 4.6; 4.7; 4.8; 4.9; 5; 5.1; 5.2; 5.3; 5.4; 5.5; 5.6; 5.7; 5.8; 5.9; 6; 6.1; 6.2; 6.3; 6.4; 6.5; 6.6; 6.7; 6.8; 6.9; 7; 7.1; 7.2; 7.3; 7.4; 7.5; 7.6; 7.7; 7.8; 7.9; 8; 8.1; 8.2; 8.3; 8.4; 8.5; 8.6; 8.7; 8.8; 8.9; 9; 9.1; 9.2; 9.3; 9.4; 9.5; 9.6; 9.7; 9.8; 9.9; 10]
  simIn.ExternalInput.any.Storage.any.Elements{16}.TimeInfo.Initialized = 1
  simIn.ExternalInput.any.Storage.any.Elements{16}.QualityInfo = tsdata.qualmetadata
  simIn.ExternalInput.any.Storage.any.Elements{16}.Data_ = [0; 0; 0; 0; 0; 0; 0; 0; 0; 0; 0; 0; 0; 0; 0; 0; 0; 0; 0; 0; 0; 0; 0; 0; 0; 0; 0; 0; 0; 0; 0; 0; 0; 0; 0; 0; 0; 0; 0; 0; 0; 0; 0; 0; 0; 0; 0; 0; 0; 0; 0; 0; 0; 0; 0; 0; 0; 0; 0; 0; 0; 0; 0; 0; 0; 0; 0; 0; 0; 0; 0; 0; 0; 0; 0; 0; 0; 0; 0; 0; 0; 0; 0; 0; 0; 0; 0; 0; 0; 0; 0; 0; 0; 0; 0; 0; 0; 0; 0; 0; 0]
  simIn.ExperimentalProperties = Simulink.Simulation.internal.ExperimentalProperties
  simIn.ModelName_ = 'ADCS_FSM_test'
  t = [0; 0.1; 0.2; 0.3; 0.4; 0.5; 0.6; 0.7; 0.8; 0.9; 1; 1.1; 1.2; 1.3; 1.4; 1.5; 1.6; 1.7; 1.8; 1.9; 2; 2.1; 2.2; 2.3; 2.4; 2.5; 2.6; 2.7; 2.8; 2.9; 3; 3.1; 3.2; 3.3; 3.4; 3.5; 3.6; 3.7; 3.8; 3.9; 4; 4.1; 4.2; 4.3; 4.4; 4.5; 4.6; 4.7; 4.8; 4.9; 5; 5.1; 5.2; 5.3; 5.4; 5.5; 5.6; 5.7; 5.8; 5.9; 6; 6.1; 6.2; 6.3; 6.4; 6.5; 6.6; 6.7; 6.8; 6.9; 7; 7.1; 7.2; 7.3; 7.4; 7.5; 7.6; 7.7; 7.8; 7.9; 8; 8.1; 8.2; 8.3; 8.4; 8.5; 8.6; 8.7; 8.8; 8.9; 9; 9.1; 9.2; 9.3; 9.4; 9.5; 9.6; 9.7; 9.8; 9.9; 10]
  u : object (value not decoded)
  y_out = [0 0 0 0 0 0 0 0]
values from neighbouring files (symbols this model uses):
  B = [1 0 0]    [parameters.m]
  h_max = 1.47    [parameters.m]
  I_RW = 1    [parameters.m]
  k_desat = 1    [parameters.m]
  kd_detumble = 1    [parameters.m]
  kd_hold = 1    [parameters.m]
  kd_point = 20    [parameters.m]
  kd_slew_fast = 1    [parameters.m]
  kd_slew_slow = 1    [parameters.m]
  kd_spin = 0    [parameters.m]
  kp_hold = 1    [parameters.m]
  kp_point = 2    [parameters.m]
  kp_slew_fast = 1    [parameters.m]
  kp_slew_slow = 1    [parameters.m]
  omega_0 = [0 0 0.0011]    [parameters.m]
  omega_ref = [0 0 0]    [parameters.m]
  P = satellite_params()    [individual_test_with_dynamics.m]    (also in parameters.m; test.m = thrusters(:, 1:3))
  q0 = [sqrt(0.5) -sqrt(0.5) 0 0]    [parameters.m]
  q_ref = [ cos(theta_ref/2) ... (first row only)    [parameters.m]
libraries: matrix_library x3, sim3dlib x2, aerolibutil x2, simulink x2
settings Model: Creator=ADMIN  LastModifiedBy=ADMIN
settings DataIOCC: ExternalInput=ds  LoadExternalInput=on

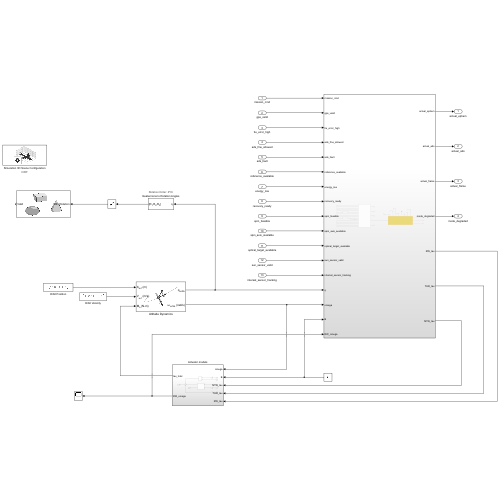
[thumbnail: Simulink's stored preview of the top-level diagram]
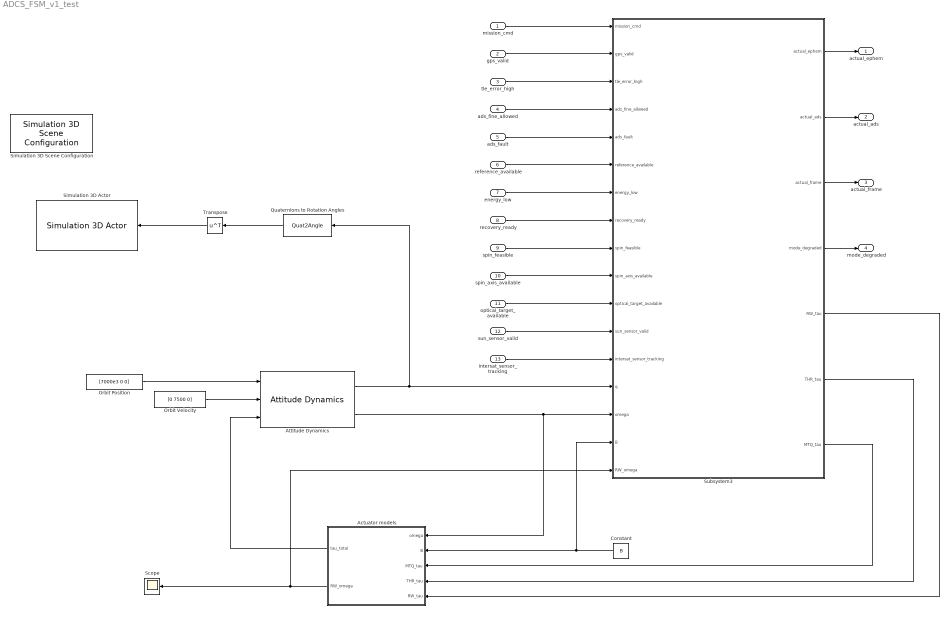
== system ADCS_FSM_v1_test ==
  mission_cmd : Inport  OutDataTypeStr=uint8  PortDimensions=1
  gps_valid : Inport  Port=2  OutDataTypeStr=boolean  PortDimensions=1
  tle_error_high : Inport  Port=3  OutDataTypeStr=boolean  PortDimensions=1
  ads_fine_allowed : Inport  Port=4  OutDataTypeStr=boolean  PortDimensions=1
  ads_fault : Inport  Port=5  OutDataTypeStr=boolean  PortDimensions=1
  reference_available : Inport  Port=6  OutDataTypeStr=boolean  PortDimensions=1
  energy_low : Inport  Port=7  OutDataTypeStr=boolean  PortDimensions=1
  recovery_ready : Inport  Port=8  OutDataTypeStr=boolean  PortDimensions=1
  spin_feasible : Inport  Port=9  OutDataTypeStr=boolean  PortDimensions=1
  spin_axis_available : Inport  Port=10  OutDataTypeStr=boolean  PortDimensions=1
  optical_target_available : Inport  Port=11  OutDataTypeStr=boolean  PortDimensions=1
  sun_sensor_valid : Inport  Port=12  OutDataTypeStr=boolean  PortDimensions=1
  intersat_sensor_tracking : Inport  Port=13  OutDataTypeStr=boolean  PortDimensions=1
  Actuator models : Subsystem
  Attitude Dynamics : AttitudeDynamics  dateOut=off  mass=P.mass0  inertia=P.I0  outputFuelStatus=off  attitude=q0.'  attitudeRate=omega_0.'  useGravGrad=off  angleUnits=Radians
  Constant : Constant  Value=B
  Orbit Position : Constant  Value=[7000e3 0 0]
  Orbit Velocity : Constant  Value=[0 7500 0]
  Quaternions to Rotation Angles : Quat2Angle
      settings: AttributesFormatString=Rotation Order: %<rotationOrder>
  Scope : Scope
      settings: ActiveDisplayYMinimum=-1  ActiveDisplayYMaximum=1
  Simulation 3D Actor : sim3dlib/Simulation 3D Actor  Priority=1  ActorName=M4V  ParentName=Scene Origin  Operation=Create at setup  InitScriptText=|  SampleTime=-1  Translation=[0 0 0]  Rotation=[0 0 0]  Scale=[1 1 1]*0.1  InputsText=M4V.Rotation  aMode=5  ActorTag=M4V  ActorType=Sim3dActor  ID=C
      | % Reserved keywords:
      | % - Actor : handle to this actor object
      | % - World : handle to the world object
      | 
      | % Examples:
      | 
      | % Create a primitive geometry (optional)
      | % createShape(Actor, 'box', [1 1 1]);
      | 
      | % Initialize values (optional)
      | % Actor.Physics = true;
      | % Actor.Color = [1 0 0];
      | M4V.Mobility = sim3d.utils.MobilityTypes.Movable;
      | 
      | % For simple motion without gravity
      | M4V.Physics = true;
      | M4V.Gravity = false;
      | M4V.Collisions = false;
  Simulation 3D Scene Configuration : sim3dlib/Simulation 3D Scene Configuration  Priority=0  ProjectFormat=Default Scenes  SceneDesc=Space  ProjectName=C:\Program Files\MATLAB\R2025b\toolbox\shared\sim3d_projects\automotive_project_windows\UE\WindowsNoEditor\VehicleSimulation.exe  ScenePath=/Game/Maps/HwStrght  EnableOpenDRIVE=off  vehTagList={'Custom';'M4V';'Scene Origin'}  vehTag=Custom  AttachedCameraRelativeTranslation=[-20000 0 0]  FreeCameraDefaultInitialTranslation=[-6, 0, 2]  AttachedCameraRelativeRotation=[0 0 0]  FreeCameraDefaultInitialRotation=[0, -15, 0]  ViewpointName=Custom  FreeCameraInitialTranslation=[-1500 0 500]  ViewpointTranslation=[0 0 0]  FreeCameraInitialRotation=[0 0 0]  ViewpointRotation=[0 0 0]  OpVisEn=off  Ts=1  EnableWindow=on  EnableRemoteAccess=off  EnableWeather=off  SunAzimuth=90  SunAltitude=40.0  EnableGeospatialSun=off  Latitude=0  Longitude=0  Date=2023-01-01  Time=10:30:00  GeoTimeZone=-5.0  SunDaylightSaving=off  wind=0  clouds=10  EnableVolumetricClouds=off  CloudCoverage=0  CloudAltitude=6  fog=0  rain=0  RaindropsEffect=off  SnowDensity=0  EnableGeospatial=off  TilesetSource=Earth terrain  UseTrueOrigin=off  OriginHeight=200  OriginLatitude=40.744652  OriginLongitude=-73.988864  MapStyle=Aerial  AdditionalAssetIDs=[]  UseAdvancedSunSky=off  SolarTime=11  TimeZone=-5  Day=21  Month=9  Year=2022  UseDaylightSavingTime=on  DSTStartDay=10  DSTStartMonth=3  DSTEndDay=3  DSTEndMonth=11  DSTSwitchHour=2  sensorTag=MainCamera1  sensorId=1  sensorName=MainCamera1  mountLoc=Origin  offsetFlag=off  tmountOffset=[0, 0, 0]  rmountOffset=[0, 0, 0]  HorizontalResolution=1280  VerticalResolution=720  HorizontalFOV=60  mountPoint=[0 0 0]  mountOrientation=[0 0 0]  aMode=0  ID=1  GeoTrigger=Inactive  ViewNameList={'Custom'}  ViewTranslationList={'[-1500 0 500]'}  ViewRotationList={'[0 0 0]'}
      settings: AttributesFormatString=ICRF  LibrarySourceBlock=aerolibsim3d/Simulation 3D Scene Configuration
  Subsystem3 : Subsystem
  Transpose : Math  Operator=transpose
  actual_ephem : Outport
  actual_ads : Outport  Port=2
  actual_frame : Outport  Port=3
  mode_degraded : Outport  Port=4
  wires:
  ads_fault/1 -> Subsystem3/5(ads_fault)
  gps_valid/1 -> Subsystem3/2(gps_valid)
  Orbit Position/1 -> Attitude Dynamics/1
  mission_cmd/1 -> Subsystem3/1(mission_cmd)
  Orbit Velocity/1 -> Attitude Dynamics/2
  tle_error_high/1 -> Subsystem3/3(tle_error_high)
  ads_fine_allowed/1 -> Subsystem3/4(ads_fine_allowed)
  reference_available/1 -> Subsystem3/6(reference_available)
  energy_low/1 -> Subsystem3/7(energy_low)
  recovery_ready/1 -> Subsystem3/8(recovery_ready)
  optical_target_available/1 -> Subsystem3/11(optical_target_available)
  spin_axis_available/1 -> Subsystem3/10(spin_axis_available)
  spin_feasible/1 -> Subsystem3/9(spin_feasible)
  sun_sensor_valid/1 -> Subsystem3/12(sun_sensor_valid)
  intersat_sensor_tracking/1 -> Subsystem3/13(intersat_sensor_tracking)
  Attitude Dynamics/2 -> Actuator models/1(omega), Subsystem3/15(omega)
  Attitude Dynamics/1 -> Quaternions to Rotation Angles/1, Subsystem3/14(q)
  Actuator models/2(RW_omega) -> Scope/1, Subsystem3/17(RW_omega)
  Subsystem3/1(actual_ephem) -> actual_ephem/1
  Subsystem3/2(actual_ads) -> actual_ads/1
  Subsystem3/3(actual_frame) -> actual_frame/1
  Subsystem3/4(mode_degraded) -> mode_degraded/1
  Subsystem3/5(RW_tau) -> Actuator models/5(RW_tau)
  Actuator models/1(tau_total) -> Attitude Dynamics/3
  Subsystem3/6(THR_tau) -> Actuator models/4(THR_tau)
  Subsystem3/7(MTQ_tau) -> Actuator models/3(MTQ_tau)
  Constant/1 -> Actuator models/2(B), Subsystem3/16(B)
  Transpose/1 -> Simulation 3D Actor/1
  Quaternions to Rotation Angles/1 -> Transpose/1

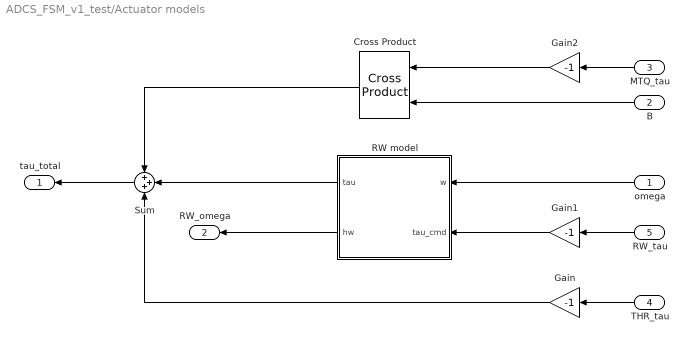
== system ADCS_FSM_v1_test/Actuator models ==
  omega : Inport
  B : Inport  Port=2
  MTQ_tau : Inport  Port=3
  THR_tau : Inport  Port=4
  RW_tau : Inport  Port=5
  Cross Product : matrix_library/Cross Product
  Gain : Gain  Gain=-1
  Gain1 : Gain  Gain=-1
  Gain2 : Gain  Gain=-1
  RW model : Subsystem
  Sum : Sum  Inputs=+++
  tau_total : Outport
  RW_omega : Outport  Port=2
  wires:
  omega/1 -> RW model/1(w)
  RW_tau/1 -> Gain1/1
  RW model/2(hw) -> RW_omega/1
  B/1 -> Cross Product/2
  MTQ_tau/1 -> Gain2/1
  Sum/1 -> tau_total/1
  Cross Product/1 -> Sum/1
  THR_tau/1 -> Gain/1
  RW model/1(tau) -> Sum/2
  Gain/1 -> Sum/3
  Gain1/1 -> RW model/2(tau_cmd)
  Gain2/1 -> Cross Product/1

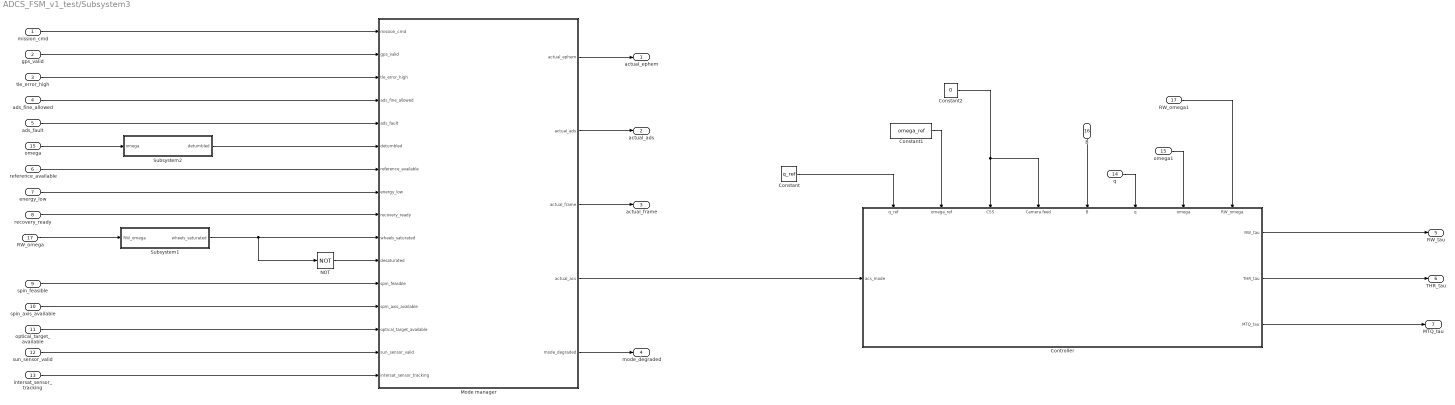
== system ADCS_FSM_v1_test/Subsystem3 ==
  mission_cmd : Inport
  gps_valid : Inport  Port=2
  tle_error_high : Inport  Port=3
  ads_fine_allowed : Inport  Port=4
  ads_fault : Inport  Port=5
  reference_available : Inport  Port=6
  energy_low : Inport  Port=7
  recovery_ready : Inport  Port=8
  spin_feasible : Inport  Port=9
  spin_axis_available : Inport  Port=10
  optical_target_available : Inport  Port=11
  sun_sensor_valid : Inport  Port=12
  intersat_sensor_tracking : Inport  Port=13
  q : Inport  Port=14
  omega : Inport  Port=15
  B : Inport  Port=16
  RW_omega : Inport  Port=17
  Constant : Constant  Value=q_ref
  Constant1 : Constant  Value=omega_ref
  Constant2 : Constant  Value=0
  Controller : Subsystem
      settings: PortSchema="{\"entries\":[{\"content\":{\"sides\":[{\"content\":{\"connectorIds\":[\"In1\"]},\"type\":\"ConnectorPlacement.EquallySpacedRectSide\",\"uuid\":\"3d0ce77c-a0dd-4e63-bb58-aa259872b360\"},{\"content\":{\"connectorIds\":[\"Out1\",\"Out2\",\"Out3\"],\"side\":\"RIGHT\"},\"type\":\"ConnectorPlacement.EquallySpacedRectSide\",\"uuid\":\"c51ce6d0-00d2-499a-9be1-102c03c9909c\"},{\"content\":{\"connectorIds\":[\"In2\",\"In3\",\"In4\",\"In5\",\"In6\",\"In7\",\"In8\",\"In9\"],\"side\":\"TOP\"},\"type\":\"ConnectorPlacement.EquallySpacedRectSide\",\"uuid\":\"ed1e7bc4-2cca-4611-893f-1128994bf2d9\"},{\"content\":{\"side\":\"BOTTOM\"},\"type\":\"ConnectorPlacement.EquallySpacedRectSide\",\"uuid\":\"574e7f6a-1005-4b0c-82f8-22f1ef6841a8\"}]},\"type\":\"ConnectorPlacement.EquallySpacedConnector\",\"uuid\":\"15c446ec-b512-4968-b865-507fd68d8b0b\"}],\"packageUris\":[\"http://schema.mathworks.com/mf0/Connector/R2020b\"],\"version\":\"1.0\"}"
  Mode manager : Subsystem
  NOT : Logic  Operator=NOT  IconShape=distinctive  AllPortsSameDT=off  OutDataTypeStr=boolean
  RW_omega1 : InportShadow  Port=17
  Subsystem1 : Subsystem
  Subsystem2 : Subsystem
  omega1 : InportShadow  Port=15
  actual_ephem : Outport
  actual_ads : Outport  Port=2
  actual_frame : Outport  Port=3
  mode_degraded : Outport  Port=4
  RW_tau : Outport  Port=5
  THR_tau : Outport  Port=6
  MTQ_tau : Outport  Port=7
  wires:
  Constant/1 -> Controller/2(q_ref)
  spin_axis_available/1 -> Mode manager/13(spin_axis_available)
  Controller/1(RW_tau) -> RW_tau/1
  Mode manager/1(actual_ephem) -> actual_ephem/1
  Mode manager/5(mode_degraded) -> mode_degraded/1
  Constant2/1 -> Controller/5(Camera feed), Controller/4(CSS)
  gps_valid/1 -> Mode manager/2(gps_valid)
  RW_omega/1 -> Subsystem1/1(RW_omega)
  Constant1/1 -> Controller/3(omega_ref)
  q/1 -> Controller/7(q)
  Subsystem2/1(detumbled) -> Mode manager/6(detumbled)
  Mode manager/2(actual_ads) -> actual_ads/1
  tle_error_high/1 -> Mode manager/3(tle_error_high)
  Controller/3(MTQ_tau) -> MTQ_tau/1
  Mode manager/4(actual_acs) -> Controller/1(acs_mode)
  Subsystem1/1(wheels_saturated) -> NOT/1, Mode manager/10(wheels_saturated)
  Mode manager/3(actual_frame) -> actual_frame/1
  sun_sensor_valid/1 -> Mode manager/15(sun_sensor_valid)
  recovery_ready/1 -> Mode manager/9(recovery_ready)
  NOT/1 -> Mode manager/11(desaturated)
  ads_fine_allowed/1 -> Mode manager/4(ads_fine_allowed)
  spin_feasible/1 -> Mode manager/12(spin_feasible)
  ads_fault/1 -> Mode manager/5(ads_fault)
  energy_low/1 -> Mode manager/8(energy_low)
  intersat_sensor_tracking/1 -> Mode manager/16(intersat_sensor_tracking)
  optical_target_available/1 -> Mode manager/14(optical_target_available)
  mission_cmd/1 -> Mode manager/1(mission_cmd)
  omega/1 -> Subsystem2/1(omega)
  reference_available/1 -> Mode manager/7(reference_available)
  Controller/2(THR_tau) -> THR_tau/1
  RW_omega1/1 -> Controller/9(RW_omega)
  omega1/1 -> Controller/8(omega)
  B/1 -> Controller/6(B)

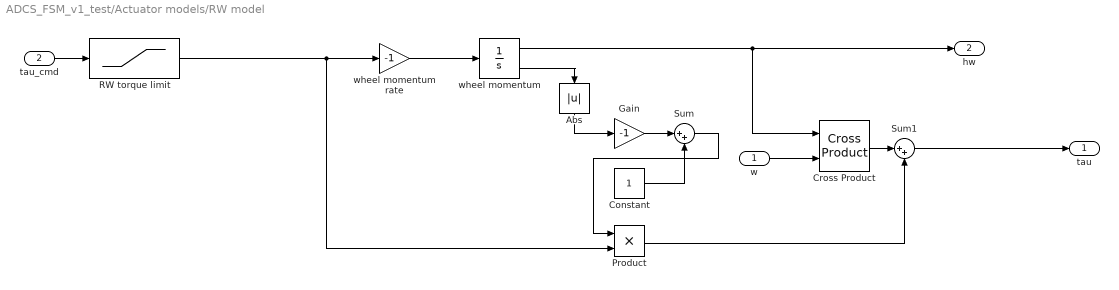
== system ADCS_FSM_v1_test/Actuator models/RW model ==
  w : Inport
  tau_cmd : Inport  Port=2
  Abs : Abs  SaturateOnIntegerOverflow=off
  Constant : Constant
  Cross Product : matrix_library/Cross Product
  Gain : Gain  Gain=-1
  Product : Product
  RW torque limit : Saturate  UpperLimit=P.rw.torque_max  LowerLimit=-P.rw.torque_max
  Sum : Sum  Inputs=|++
  Sum1 : Sum  Inputs=|++
  wheel momentum : Integrator  InitialCondition=[0 0 0]  LimitOutput=on  UpperSaturationLimit=P.rw.h_max  LowerSaturationLimit=-P.rw.h_max  ShowSaturationPort=on
  wheel momentum rate : Gain  Gain=-1
  tau : Outport
  hw : Outport  Port=2
  wires:
  Abs/1 -> Gain/1
  wheel momentum rate/1 -> wheel momentum/1
  RW torque limit/1 -> Product/2, wheel momentum rate/1
  wheel momentum/1 -> Cross Product/1, hw/1
  wheel momentum/2 -> Abs/1
  Gain/1 -> Sum/1
  Constant/1 -> Sum/2
  Sum/1 -> Product/1
  tau_cmd/1 -> RW torque limit/1
  Product/1 -> Sum1/2
  w/1 -> Cross Product/2
  Cross Product/1 -> Sum1/1
  Sum1/1 -> tau/1

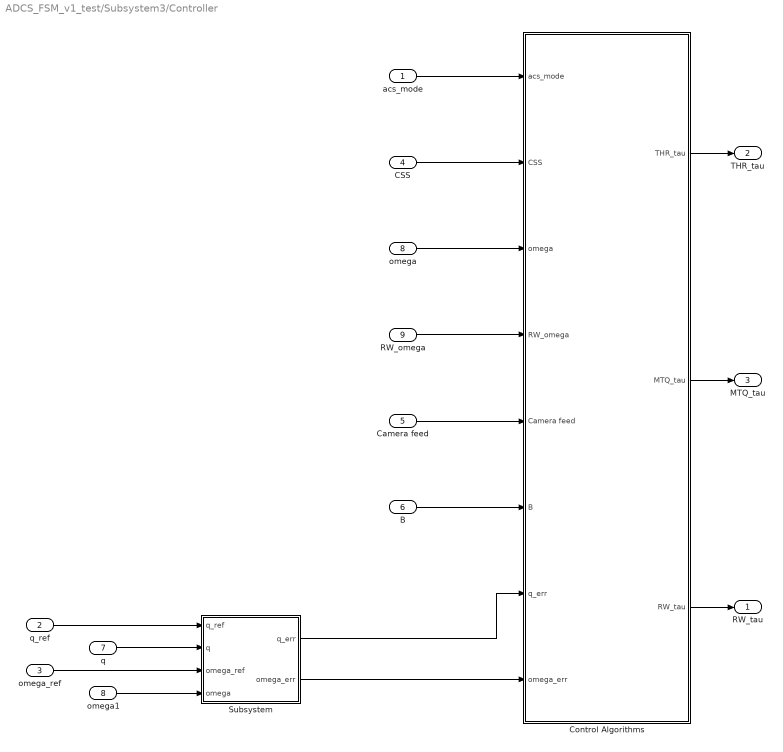
== system ADCS_FSM_v1_test/Subsystem3/Controller ==
  acs_mode : Inport
  q_ref : Inport  Port=2
  omega_ref : Inport  Port=3
  CSS : Inport  Port=4
  Camera feed : Inport  Port=5
  B : Inport  Port=6
  q : Inport  Port=7
  omega : Inport  Port=8
  RW_omega : Inport  Port=9
  Control Algorithms : Subsystem
  Subsystem : Subsystem
  omega1 : InportShadow  Port=8
  RW_tau : Outport
  THR_tau : Outport  Port=2
  MTQ_tau : Outport  Port=3
  wires:
  Subsystem/1(q_err) -> Control Algorithms/7(q_err)
  RW_omega/1 -> Control Algorithms/4(RW_omega)
  CSS/1 -> Control Algorithms/2(CSS)
  Camera feed/1 -> Control Algorithms/5(Camera feed)
  omega/1 -> Control Algorithms/3(omega)
  B/1 -> Control Algorithms/6(B)
  Subsystem/2(omega_err) -> Control Algorithms/8(omega_err)
  Control Algorithms/1(THR_tau) -> THR_tau/1
  Control Algorithms/2(MTQ_tau) -> MTQ_tau/1
  Control Algorithms/3(RW_tau) -> RW_tau/1
  q_ref/1 -> Subsystem/1(q_ref)
  q/1 -> Subsystem/2(q)
  omega_ref/1 -> Subsystem/3(omega_ref)
  omega1/1 -> Subsystem/4(omega)
  acs_mode/1 -> Control Algorithms/1(acs_mode)

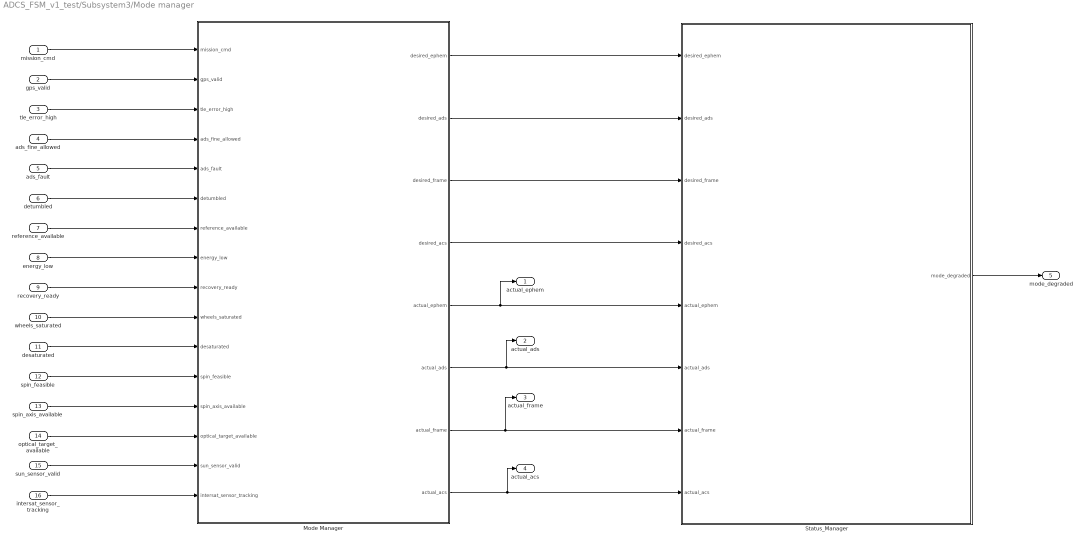
== system ADCS_FSM_v1_test/Subsystem3/Mode manager ==
  mission_cmd : Inport
  gps_valid : Inport  Port=2
  tle_error_high : Inport  Port=3
  ads_fine_allowed : Inport  Port=4
  ads_fault : Inport  Port=5
  detumbled : Inport  Port=6
  reference_available : Inport  Port=7
  energy_low : Inport  Port=8
  recovery_ready : Inport  Port=9
  wheels_saturated : Inport  Port=10
  desaturated : Inport  Port=11
  spin_feasible : Inport  Port=12
  spin_axis_available : Inport  Port=13
  optical_target_available : Inport  Port=14
  sun_sensor_valid : Inport  Port=15
  intersat_sensor_tracking : Inport  Port=16
  Mode Manager : Subsystem
  Status_Manager : Stateflow chart  TreatAsAtomicUnit=on
  actual_ephem : Outport
  actual_ads : Outport  Port=2
  actual_frame : Outport  Port=3
  actual_acs : Outport  Port=4
  mode_degraded : Outport  Port=5
  wires:
  recovery_ready/1 -> Mode Manager/9(recovery_ready)
  Mode Manager/2(desired_ads) -> Status_Manager/2(desired_ads)
  Mode Manager/8(actual_acs) -> actual_acs/1, Status_Manager/8(actual_acs)
  Mode Manager/1(desired_ephem) -> Status_Manager/1(desired_ephem)
  Mode Manager/5(actual_ephem) -> actual_ephem/1, Status_Manager/5(actual_ephem)
  Mode Manager/6(actual_ads) -> actual_ads/1, Status_Manager/6(actual_ads)
  Mode Manager/7(actual_frame) -> actual_frame/1, Status_Manager/7(actual_frame)
  Mode Manager/3(desired_frame) -> Status_Manager/3(desired_frame)
  Mode Manager/4(desired_acs) -> Status_Manager/4(desired_acs)
  reference_available/1 -> Mode Manager/7(reference_available)
  mission_cmd/1 -> Mode Manager/1(mission_cmd)
  ads_fault/1 -> Mode Manager/5(ads_fault)
  ads_fine_allowed/1 -> Mode Manager/4(ads_fine_allowed)
  wheels_saturated/1 -> Mode Manager/10(wheels_saturated)
  optical_target_available/1 -> Mode Manager/14(optical_target_available)
  detumbled/1 -> Mode Manager/6(detumbled)
  intersat_sensor_tracking/1 -> Mode Manager/16(intersat_sensor_tracking)
  desaturated/1 -> Mode Manager/11(desaturated)
  spin_feasible/1 -> Mode Manager/12(spin_feasible)
  tle_error_high/1 -> Mode Manager/3(tle_error_high)
  energy_low/1 -> Mode Manager/8(energy_low)
  Status_Manager/1(mode_degraded) -> mode_degraded/1
  spin_axis_available/1 -> Mode Manager/13(spin_axis_available)
  sun_sensor_valid/1 -> Mode Manager/15(sun_sensor_valid)
  gps_valid/1 -> Mode Manager/2(gps_valid)

== system ADCS_FSM_v1_test/Subsystem3/Subsystem1 ==
  RW_omega : Inport
  Abs : Abs  SaturateOnIntegerOverflow=off
  Compare To Constant : simulink/Logic and Bit Operations/Compare To Constant  relop=<=  const=h_max  OutDataTypeStr=boolean
  Gain : Gain  Gain=I_RW
  Max of Elements : MinMax  Function=max
  wheels_saturated : Outport
  wires:
  Gain/1 -> Compare To Constant/1
  Abs/1 -> Max of Elements/1
  RW_omega/1 -> Abs/1
  Max of Elements/1 -> Gain/1
  Compare To Constant/1 -> wheels_saturated/1

== system ADCS_FSM_v1_test/Subsystem3/Subsystem2 ==
  omega : Inport
  Compare To Constant : simulink/Logic and Bit Operations/Compare To Constant  relop=<=  const=omega_thr^2  OutDataTypeStr=boolean
  Dot Product : DotProduct  OutDataTypeStr=Inherit: Inherit via internal rule
  detumbled : Outport
  wires:
  Compare To Constant/1 -> detumbled/1
  omega/1 -> Dot Product/2, Dot Product/1
  Dot Product/1 -> Compare To Constant/1

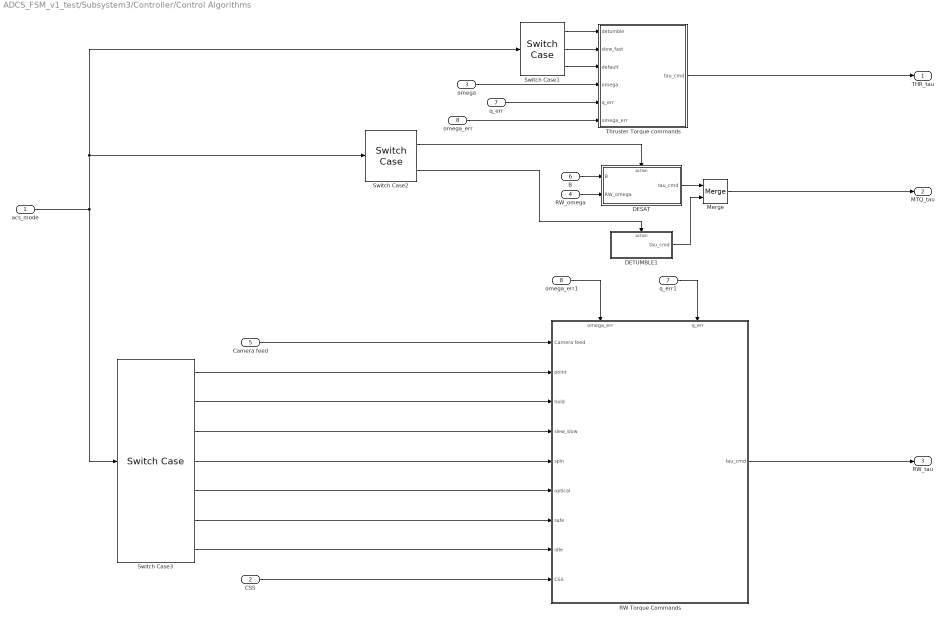
== system ADCS_FSM_v1_test/Subsystem3/Controller/Control Algorithms ==
  acs_mode : Inport
  CSS : Inport  Port=2
  omega : Inport  Port=3
  RW_omega : Inport  Port=4
  Camera feed : Inport  Port=5
  B : Inport  Port=6
  q_err : Inport  Port=7
  omega_err : Inport  Port=8
  DESAT : Subsystem  TreatAsAtomicUnit=on
  DETUMBLE1 : Subsystem  TreatAsAtomicUnit=on
  Merge : Merge
  RW Torque Commands : Subsystem
      settings: PortSchema="{\"entries\":[{\"content\":{\"sides\":[{\"content\":{\"connectorIds\":[\"In1\",\"In2\",\"In3\",\"In4\",\"In5\",\"In6\",\"In7\",\"In8\",\"In9\"]},\"type\":\"ConnectorPlacement.EquallySpacedRectSide\",\"uuid\":\"3d0ce77c-a0dd-4e63-bb58-aa259872b360\"},{\"content\":{\"connectorIds\":[\"Out1\"],\"side\":\"RIGHT\"},\"type\":\"ConnectorPlacement.EquallySpacedRectSide\",\"uuid\":\"c51ce6d0-00d2-499a-9be1-102c03c9909c\"},{\"content\":{\"connectorIds\":[\"In10\",\"In11\"],\"side\":\"TOP\"},\"type\":\"ConnectorPlacement.EquallySpacedRectSide\",\"uuid\":\"ed1e7bc4-2cca-4611-893f-1128994bf2d9\"}]},\"type\":\"ConnectorPlacement.EquallySpacedConnector\",\"uuid\":\"15c446ec-b512-4968-b865-507fd68d8b0b\"}],\"packageUris\":[\"http://schema.mathworks.com/mf0/Connector/R2020b\"],\"version\":\"1.0\"}"
  Switch Case1 : SwitchCase  CaseConditions={1,5}
  Switch Case2 : SwitchCase  CaseConditions={7}
  Switch Case3 : SwitchCase  CaseConditions={2,3,4,6,8,9}
  Thruster Torque commands : Subsystem
  omega_err1 : InportShadow  Port=8
  q_err1 : InportShadow  Port=7
  THR_tau : Outport
  MTQ_tau : Outport  Port=2
  RW_tau : Outport  Port=3
  wires:
  Camera feed/1 -> RW Torque Commands/1(Camera feed)
  RW_omega/1 -> DESAT/2(RW_omega)
  B/1 -> DESAT/1(B)
  RW Torque Commands/1(tau_cmd) -> RW_tau/1
  CSS/1 -> RW Torque Commands/9(CSS)
  Thruster Torque commands/1(tau_cmd) -> THR_tau/1
  omega/1 -> Thruster Torque commands/4(omega)
  omega_err/1 -> Thruster Torque commands/6(omega_err)
  q_err/1 -> Thruster Torque commands/5(q_err)
  omega_err1/1 -> RW Torque Commands/10(omega_err)
  q_err1/1 -> RW Torque Commands/11(q_err)
  Switch Case1/1 -> Thruster Torque commands/1(detumble)
  Switch Case1/2 -> Thruster Torque commands/2(slew_fast)
  Switch Case1/3 -> Thruster Torque commands/3(default)
  DETUMBLE1/1(tau_cmd) -> Merge/2
  Switch Case2/2 -> DETUMBLE1/Action
  DESAT/1(tau_cmd) -> Merge/1
  Merge/1 -> MTQ_tau/1
  Switch Case2/1 -> DESAT/Action
  Switch Case3/1 -> RW Torque Commands/2(point)
  Switch Case3/2 -> RW Torque Commands/3(hold)
  Switch Case3/3 -> RW Torque Commands/4(slew_slow)
  Switch Case3/4 -> RW Torque Commands/5(spin)
  Switch Case3/5 -> RW Torque Commands/6(optical)
  Switch Case3/6 -> RW Torque Commands/7(safe)
  Switch Case3/7 -> RW Torque Commands/8(idle)
  acs_mode/1 -> Switch Case3/1, Switch Case2/1, Switch Case1/1

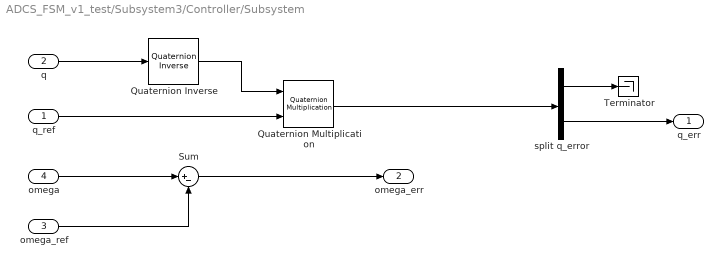
== system ADCS_FSM_v1_test/Subsystem3/Controller/Subsystem ==
  q_ref : Inport
  q : Inport  Port=2
  omega_ref : Inport  Port=3
  omega : Inport  Port=4
  Quaternion Inverse : aerolibutil/Quaternion Inverse
  Quaternion Multiplication : aerolibutil/Quaternion Multiplication
  Sum : Sum  Inputs=|+-
  Terminator : Terminator
  split q_error : Demux  Outputs=[1 3]
  q_err : Outport
  omega_err : Outport  Port=2
  wires:
  q/1 -> Quaternion Inverse/1
  Sum/1 -> omega_err/1
  Quaternion Multiplication/1 -> split q_error/1
  split q_error/2 -> q_err/1
  split q_error/1 -> Terminator/1
  q_ref/1 -> Quaternion Multiplication/2
  Quaternion Inverse/1 -> Quaternion Multiplication/1
  omega/1 -> Sum/1
  omega_ref/1 -> Sum/2

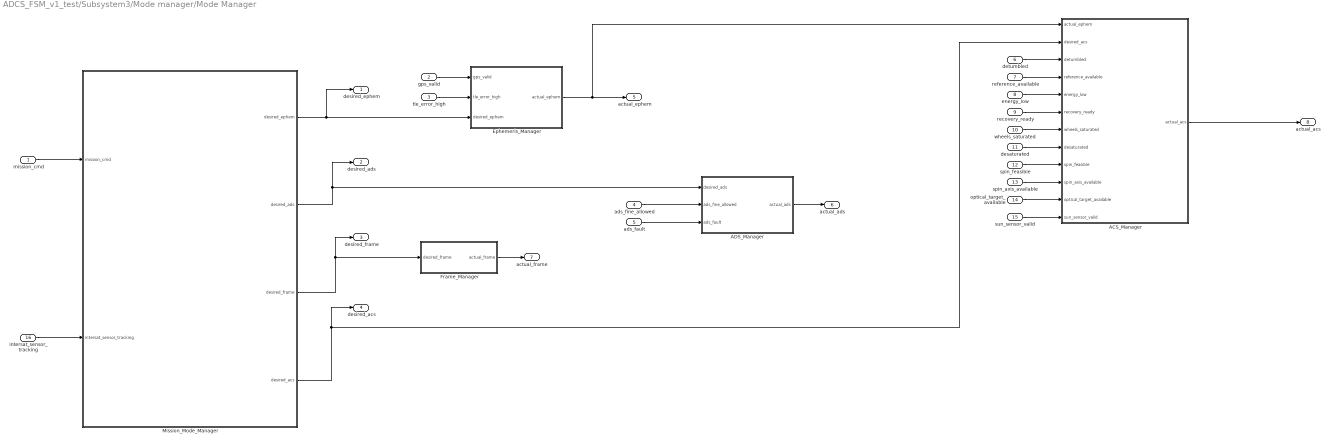
== system ADCS_FSM_v1_test/Subsystem3/Mode manager/Mode Manager ==
  mission_cmd : Inport  OutDataTypeStr=uint8  PortDimensions=1
  gps_valid : Inport  Port=2  OutDataTypeStr=boolean  PortDimensions=1
  tle_error_high : Inport  Port=3  OutDataTypeStr=boolean  PortDimensions=1
  ads_fine_allowed : Inport  Port=4  OutDataTypeStr=boolean  PortDimensions=1
  ads_fault : Inport  Port=5  OutDataTypeStr=boolean  PortDimensions=1
  detumbled : Inport  Port=6  OutDataTypeStr=boolean  PortDimensions=1
  reference_available : Inport  Port=7  OutDataTypeStr=boolean  PortDimensions=1
  energy_low : Inport  Port=8  OutDataTypeStr=boolean  PortDimensions=1
  recovery_ready : Inport  Port=9  OutDataTypeStr=boolean  PortDimensions=1
  wheels_saturated : Inport  Port=10  OutDataTypeStr=boolean  PortDimensions=1
  desaturated : Inport  Port=11  OutDataTypeStr=boolean  PortDimensions=1
  spin_feasible : Inport  Port=12  OutDataTypeStr=boolean  PortDimensions=1
  spin_axis_available : Inport  Port=13  OutDataTypeStr=boolean  PortDimensions=1
  optical_target_available : Inport  Port=14  OutDataTypeStr=boolean  PortDimensions=1
  sun_sensor_valid : Inport  Port=15  OutDataTypeStr=boolean  PortDimensions=1
  intersat_sensor_tracking : Inport  Port=16  OutDataTypeStr=boolean  PortDimensions=1
  ACS_Manager : Stateflow chart  TreatAsAtomicUnit=on
      settings: PortSchema="{\"entries\":[{\"content\":{\"sides\":[{\"content\":{\"connectorIds\":[\"In2\",\"In1\",\"In3\",\"In4\",\"In5\",\"In6\",\"In7\",\"In8\",\"In9\",\"In10\",\"In11\",\"In12\"]},\"type\":\"ConnectorPlacement.EquallySpacedRectSide\",\"uuid\":\"c64f5ed7-7a07-4761-a251-d625087249f8\"},{\"content\":{\"connectorIds\":[\"Out1\"],\"side\":\"RIGHT\"},\"type\":\"ConnectorPlacement.EquallySpacedRectSide\",\"uuid\":\"ff17dfa7-5a32-4799-bec0-131df3b46d45\"},{\"content\":{\"side\":\"TOP\"},\"type\":\"ConnectorPlacement.EquallySpacedRectSide\",\"uuid\":\"acaf274e-12ec-4fab-ab7e-ad580afcef6e\"}]},\"type\":\"ConnectorPlacement.EquallySpacedConnector\",\"uuid\":\"7d19de63-b993-417e-b6e9-9dc888da130b\"}],\"packageUris\":[\"http://schema.mathworks.com/mf0/Connector/R2020b\"],\"version\":\"1.0\"}"
  ADS_Manager : Stateflow chart  TreatAsAtomicUnit=on
  Ephemeris_Manager : Stateflow chart  TreatAsAtomicUnit=on
      settings: PortSchema="{\"entries\":[{\"content\":{\"sides\":[{\"content\":{\"connectorIds\":[\"In2\",\"In3\",\"In1\"]},\"type\":\"ConnectorPlacement.EquallySpacedRectSide\",\"uuid\":\"cbbccf67-8c60-498d-a98a-76db8747fb3a\"},{\"content\":{\"connectorIds\":[\"Out1\"],\"side\":\"RIGHT\"},\"type\":\"ConnectorPlacement.EquallySpacedRectSide\",\"uuid\":\"743b35d2-d398-4833-9c20-93b5e77612f2\"},{\"content\":{\"side\":\"TOP\"},\"type\":\"ConnectorPlacement.EquallySpacedRectSide\",\"uuid\":\"56075cc1-c683-438a-85bf-78d94186ffa6\"}]},\"type\":\"ConnectorPlacement.EquallySpacedConnector\",\"uuid\":\"bae867d4-09fc-4097-a23b-eff5fb3633ac\"}],\"packageUris\":[\"http://schema.mathworks.com/mf0/Connector/R2020b\"],\"version\":\"1.0\"}"
  Frame_Manager : Stateflow chart  TreatAsAtomicUnit=on
  Mission_Mode_Manager : Stateflow chart  TreatAsAtomicUnit=on
  desired_ephem : Outport
  desired_ads : Outport  Port=2
  desired_frame : Outport  Port=3
  desired_acs : Outport  Port=4
  actual_ephem : Outport  Port=5
  actual_ads : Outport  Port=6
  actual_frame : Outport  Port=7
  actual_acs : Outport  Port=8
  wires:
  sun_sensor_valid/1 -> ACS_Manager/12(sun_sensor_valid)
  ACS_Manager/1(actual_acs) -> actual_acs/1
  Mission_Mode_Manager/4(desired_acs) -> ACS_Manager/1(desired_acs), desired_acs/1
  energy_low/1 -> ACS_Manager/5(energy_low)
  Mission_Mode_Manager/1(desired_ephem) -> Ephemeris_Manager/1(desired_ephem), desired_ephem/1
  Frame_Manager/1(actual_frame) -> actual_frame/1
  optical_target_available/1 -> ACS_Manager/11(optical_target_available)
  Mission_Mode_Manager/2(desired_ads) -> desired_ads/1, ADS_Manager/1(desired_ads)
  tle_error_high/1 -> Ephemeris_Manager/3(tle_error_high)
  reference_available/1 -> ACS_Manager/4(reference_available)
  detumbled/1 -> ACS_Manager/3(detumbled)
  wheels_saturated/1 -> ACS_Manager/7(wheels_saturated)
  Mission_Mode_Manager/3(desired_frame) -> desired_frame/1, Frame_Manager/1(desired_frame)
  ADS_Manager/1(actual_ads) -> actual_ads/1
  ads_fine_allowed/1 -> ADS_Manager/2(ads_fine_allowed)
  Ephemeris_Manager/1(actual_ephem) -> actual_ephem/1, ACS_Manager/2(actual_ephem)
  gps_valid/1 -> Ephemeris_Manager/2(gps_valid)
  intersat_sensor_tracking/1 -> Mission_Mode_Manager/2(intersat_sensor_tracking)
  ads_fault/1 -> ADS_Manager/3(ads_fault)
  recovery_ready/1 -> ACS_Manager/6(recovery_ready)
  mission_cmd/1 -> Mission_Mode_Manager/1(mission_cmd)
  spin_axis_available/1 -> ACS_Manager/10(spin_axis_available)
  desaturated/1 -> ACS_Manager/8(desaturated)
  spin_feasible/1 -> ACS_Manager/9(spin_feasible)

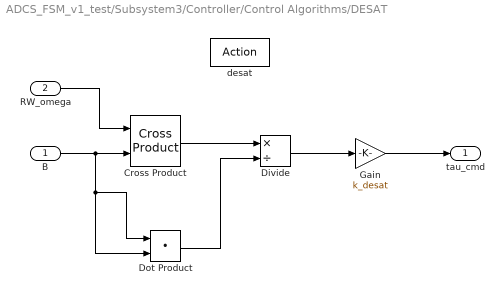
== system ADCS_FSM_v1_test/Subsystem3/Controller/Control Algorithms/DESAT ==
  B : Inport
  RW_omega : Inport  Port=2
  desat : ActionPort  ActionPortLabel=case [ 7 ]:
  Cross Product : matrix_library/Cross Product
  Divide : Product  Inputs=*/
  Dot Product : DotProduct  OutDataTypeStr=Inherit: Inherit via internal rule
  Gain : Gain  Gain=k_desat
  tau_cmd : Outport
  wires:
  B/1 -> Dot Product/1, Dot Product/2, Cross Product/2
  Divide/1 -> Gain/1
  Gain/1 -> tau_cmd/1
  Cross Product/1 -> Divide/1
  RW_omega/1 -> Cross Product/1
  Dot Product/1 -> Divide/2

== system ADCS_FSM_v1_test/Subsystem3/Controller/Control Algorithms/DETUMBLE1 ==
  detumble : ActionPort  ActionPortLabel=default:
  Constant : Constant  Value=[0 0 0]
  tau_cmd : Outport
  wires:
  Constant/1 -> tau_cmd/1

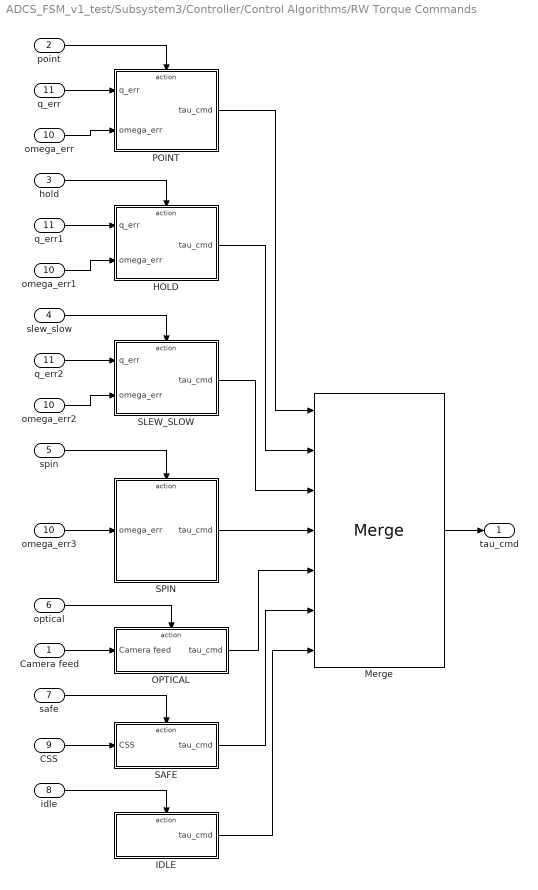
== system ADCS_FSM_v1_test/Subsystem3/Controller/Control Algorithms/RW Torque Commands ==
  Camera feed : Inport
  point : Inport  Port=2
  hold : Inport  Port=3
  slew_slow : Inport  Port=4
  spin : Inport  Port=5
  optical : Inport  Port=6
  safe : Inport  Port=7
  idle : Inport  Port=8
  CSS : Inport  Port=9
  omega_err : Inport  Port=10
  q_err : Inport  Port=11
  HOLD : Subsystem  TreatAsAtomicUnit=on
  IDLE : Subsystem  TreatAsAtomicUnit=on
  Merge : Merge  Inputs=7
  OPTICAL : Subsystem  TreatAsAtomicUnit=on
  POINT : Subsystem  TreatAsAtomicUnit=on
  SAFE : Subsystem  TreatAsAtomicUnit=on
  SLEW_SLOW : Subsystem  TreatAsAtomicUnit=on
  SPIN : Subsystem  TreatAsAtomicUnit=on
  omega_err1 : InportShadow  Port=10
  omega_err2 : InportShadow  Port=10
  omega_err3 : InportShadow  Port=10
  q_err1 : InportShadow  Port=11
  q_err2 : InportShadow  Port=11
  tau_cmd : Outport
  wires:
  safe/1 -> SAFE/Action
  slew_slow/1 -> SLEW_SLOW/Action
  hold/1 -> HOLD/Action
  SLEW_SLOW/1(tau_cmd) -> Merge/3
  point/1 -> POINT/Action
  q_err1/1 -> HOLD/1(q_err)
  omega_err/1 -> POINT/2(omega_err)
  q_err/1 -> POINT/1(q_err)
  omega_err1/1 -> HOLD/2(omega_err)
  q_err2/1 -> SLEW_SLOW/1(q_err)
  omega_err2/1 -> SLEW_SLOW/2(omega_err)
  spin/1 -> SPIN/Action
  omega_err3/1 -> SPIN/1(omega_err)
  optical/1 -> OPTICAL/Action
  Camera feed/1 -> OPTICAL/1(Camera feed)
  CSS/1 -> SAFE/1(CSS)
  idle/1 -> IDLE/Action
  POINT/1(tau_cmd) -> Merge/1
  HOLD/1(tau_cmd) -> Merge/2
  SPIN/1(tau_cmd) -> Merge/4
  OPTICAL/1(tau_cmd) -> Merge/5
  SAFE/1(tau_cmd) -> Merge/6
  IDLE/1(tau_cmd) -> Merge/7
  Merge/1 -> tau_cmd/1

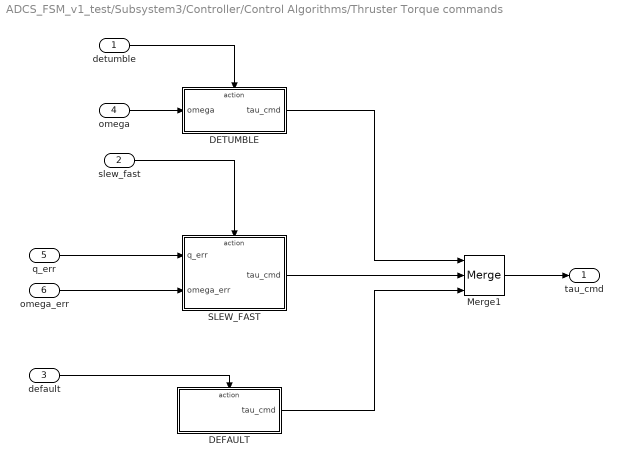
== system ADCS_FSM_v1_test/Subsystem3/Controller/Control Algorithms/Thruster Torque commands ==
  detumble : Inport
  slew_fast : Inport  Port=2
  default : Inport  Port=3
  omega : Inport  Port=4
  q_err : Inport  Port=5
  omega_err : Inport  Port=6
  DEFAULT : Subsystem  TreatAsAtomicUnit=on
  DETUMBLE : Subsystem  TreatAsAtomicUnit=on
  Merge1 : Merge  Inputs=3
  SLEW_FAST : Subsystem  TreatAsAtomicUnit=on
  tau_cmd : Outport
  wires:
  SLEW_FAST/1(tau_cmd) -> Merge1/2
  omega/1 -> DETUMBLE/1(omega)
  DETUMBLE/1(tau_cmd) -> Merge1/1
  DEFAULT/1(tau_cmd) -> Merge1/3
  Merge1/1 -> tau_cmd/1
  q_err/1 -> SLEW_FAST/1(q_err)
  omega_err/1 -> SLEW_FAST/2(omega_err)
  slew_fast/1 -> SLEW_FAST/Action
  detumble/1 -> DETUMBLE/Action
  default/1 -> DEFAULT/Action

== system ADCS_FSM_v1_test/Subsystem3/Controller/Control Algorithms/RW Torque Commands/HOLD ==
  q_err : Inport
  omega_err : Inport  Port=2
  hold : ActionPort  ActionPortLabel=case [ 3 ]:
  Gain : Gain  Gain=kd_hold
  Gain1 : Gain  Gain=kp_hold
  Sum : Sum  Inputs=|++
  tau_cmd : Outport
  wires:
  q_err/1 -> Gain1/1
  Gain1/1 -> Sum/1
  Sum/1 -> tau_cmd/1
  omega_err/1 -> Gain/1
  Gain/1 -> Sum/2

== system ADCS_FSM_v1_test/Subsystem3/Controller/Control Algorithms/RW Torque Commands/IDLE ==
  idle : ActionPort  ActionPortLabel=default:
  Constant : Constant  Value=[0 0 0]
  tau_cmd : Outport
  wires:
  Constant/1 -> tau_cmd/1

== system ADCS_FSM_v1_test/Subsystem3/Controller/Control Algorithms/RW Torque Commands/OPTICAL ==
  Camera feed : Inport
  optical : ActionPort  ActionPortLabel=case [ 8 ]:
  Constant : Constant  Value=[0 0 0]
  tau_cmd : Outport
  wires:
  Constant/1 -> tau_cmd/1

== system ADCS_FSM_v1_test/Subsystem3/Controller/Control Algorithms/RW Torque Commands/POINT ==
  q_err : Inport
  omega_err : Inport  Port=2
  point : ActionPort  ActionPortLabel=case [ 2 ]:
  Gain : Gain  Gain=kd_point
  Gain1 : Gain  Gain=kp_point
  Sum : Sum  Inputs=|++
  tau_cmd : Outport
  wires:
  Sum/1 -> tau_cmd/1
  omega_err/1 -> Gain/1
  q_err/1 -> Gain1/1
  Gain1/1 -> Sum/1
  Gain/1 -> Sum/2

== system ADCS_FSM_v1_test/Subsystem3/Controller/Control Algorithms/RW Torque Commands/SAFE ==
  CSS : Inport
  safe : ActionPort  ActionPortLabel=case [ 9 ]:
  Constant : Constant  Value=[0 0 0]
  tau_cmd : Outport
  wires:
  Constant/1 -> tau_cmd/1

== system ADCS_FSM_v1_test/Subsystem3/Controller/Control Algorithms/RW Torque Commands/SLEW_SLOW ==
  q_err : Inport
  omega_err : Inport  Port=2
  slew_slow : ActionPort  ActionPortLabel=case [ 4 ]:
  Gain : Gain  Gain=kd_slew_slow
  Gain1 : Gain  Gain=kp_slew_slow
  Sum : Sum  Inputs=|++
  tau_cmd : Outport
  wires:
  Gain/1 -> Sum/2
  omega_err/1 -> Gain/1
  Sum/1 -> tau_cmd/1
  Gain1/1 -> Sum/1
  q_err/1 -> Gain1/1

== system ADCS_FSM_v1_test/Subsystem3/Controller/Control Algorithms/RW Torque Commands/SPIN ==
  omega_err : Inport
  spin : ActionPort  ActionPortLabel=case [ 6 ]:
  Gain : Gain  Gain=kd_spin
  tau_cmd : Outport
  wires:
  Gain/1 -> tau_cmd/1
  omega_err/1 -> Gain/1

== system ADCS_FSM_v1_test/Subsystem3/Controller/Control Algorithms/Thruster Torque commands/DEFAULT ==
  default : ActionPort  ActionPortLabel=default:
  Constant : Constant  Value=[0 0 0]
  tau_cmd : Outport
  wires:
  Constant/1 -> tau_cmd/1

== system ADCS_FSM_v1_test/Subsystem3/Controller/Control Algorithms/Thruster Torque commands/DETUMBLE ==
  omega : Inport
  detumble : ActionPort  ActionPortLabel=case [ 1 ]:
  Gain : Gain  Gain=kd_detumble
  tau_cmd : Outport
  wires:
  omega/1 -> Gain/1
  Gain/1 -> tau_cmd/1

== system ADCS_FSM_v1_test/Subsystem3/Controller/Control Algorithms/Thruster Torque commands/SLEW_FAST ==
  q_err : Inport
  omega_err : Inport  Port=2
  slew_fast : ActionPort  ActionPortLabel=case [ 5 ]:
  Gain : Gain  Gain=kd_slew_fast
  Gain1 : Gain  Gain=kp_slew_fast
  Sum : Sum  Inputs=|++
  tau_cmd : Outport
  wires:
  Gain/1 -> Sum/2
  omega_err/1 -> Gain/1
  Sum/1 -> tau_cmd/1
  Gain1/1 -> Sum/1
  q_err/1 -> Gain1/1

== stateflow chart ADCS_FSM_v1_test/Subsystem3/Mode manager/Mode Manager/Frame_Manager ==
  state FRAME_INERTIAL
    entry:
    actual_frame = uint8(2);
  state FRAME_LVLH
    entry:
    actual_frame = uint8(3);
  state FRAME_BODY
    entry:
    actual_frame = uint8(1);
  state FRAME_EARTH_TARGET
    entry:
    actual_frame = uint8(4);
  state FRAME_IDLE
    entry:
    actual_frame = uint8(0);
  state FRAME_IMAGING_TDI
    entry:
    actual_frame = uint8(6);
  state FRAME_VNB
    entry:
    actual_frame = uint8(5);
  FRAME_INERTIAL -> (junction 11) : [desired_frame ~= uint8(2)]
  (junction 11) -> FRAME_INERTIAL [order 3] : [desired_frame == uint8(2)]
  FRAME_LVLH -> (junction 11) : [desired_frame ~= uint8(3)]
  (junction 11) -> FRAME_LVLH [order 4] : [desired_frame == uint8(3)]
  FRAME_BODY -> (junction 11) : [desired_frame ~= uint8(1)]
  (junction 11) -> FRAME_BODY [order 2] : [desired_frame == uint8(1)]
  FRAME_EARTH_TARGET -> (junction 11) : [desired_frame ~= uint8(4)]
  (junction 11) -> FRAME_EARTH_TARGET [order 5] : [desired_frame == uint8(4)]
  (junction 11) -> FRAME_IDLE [order 1] : [desired_frame == uint8(0)]
  FRAME_IDLE -> (junction 11) : [desired_frame ~= uint8(0)]
  FRAME_IMAGING_TDI -> (junction 11) : [desired_frame ~= uint8(6)]
  (junction 11) -> FRAME_VNB [order 6] : [desired_frame == uint8(5)]
  (junction 11) -> FRAME_IMAGING_TDI [order 7] : [desired_frame == uint8(6)]
  FRAME_VNB -> (junction 11) : [desired_frame ~= uint8(5)]
  (default) -> FRAME_IDLE
  data: desired_frame input uint8; actual_frame output uint8 =0

== stateflow chart ADCS_FSM_v1_test/Subsystem3/Mode manager/Mode Manager/ACS_Manager ==
  state ACS_DETUMBLE
    entry:
    actual_acs = uint8(1);
  state ACS_POINT
    entry:
    actual_acs = uint8(2);
  state ACS_IDLE
    entry:
    actual_acs = uint8(0);
  state ACS_SLEW_SLOW
    entry:
    actual_acs = uint8(4);
  state ACS_DESAT
    entry:
    actual_acs = uint8(7);
    %exit:
    %desaturated = 1;
  state ACS_HOLD
    entry:
    actual_acs = uint8(3);
  state ACS_OPTICAL
    entry:
    actual_acs = uint8(8);
  state ACS_SPIN
    entry:
    actual_acs = uint8(6);
  state ACS_SLEW_FAST
    entry:
    actual_acs = uint8(5);
  state ACS_SAFE
    entry:
    actual_acs = uint8(9);
  ACS_SLEW_SLOW -> ACS_DESAT [order 3] : [wheels_saturated && ~energy_low]
  ACS_OPTICAL -> ACS_POINT [order 3] : [~optical_target_available &&...
      |  ~energy_low]
  (junction 25) -> ACS_DETUMBLE [order 2] : [desired_acs == uint8(1)]
  ACS_DETUMBLE -> (junction 25) : [desired_acs ~= uint8(1)]
  ACS_POINT -> ACS_SAFE [order 2] : [energy_low || ~reference_available ||...
      |  ~detumbled || actual_ephem == uint8(0)]
  (junction 25) -> ACS_IDLE [order 1] : [desired_acs == uint8(0)]
  ACS_POINT -> (junction 25) [order 1] : [desired_acs ~= uint8(2) &&...
      |  ~(desired_acs == uint8(8) &&...
      |  ~optical_target_available)]
  (junction 25) -> ACS_POINT [order 3] : [desired_acs == uint8(2)]
  (default) -> ACS_IDLE
  ACS_IDLE -> (junction 25) : [desired_acs ~= uint8(0)]
  (junction 25) -> ACS_SLEW_SLOW [order 5] : [desired_acs == uint8(4)]
  ACS_SLEW_SLOW -> (junction 25) [order 1] : [desired_acs ~= uint8(4)]
  ACS_SLEW_SLOW -> ACS_SAFE [order 2] : [energy_low || ~detumbled ||...
      |  actual_ephem == uint8(0)]
  ACS_HOLD -> (junction 25) [order 1] : [desired_acs ~= uint8(3)]
  ACS_DESAT -> (junction 25) [order 1] : [desired_acs ~= uint8(7) &&...
      |  desaturated && recovery_ready &&...
      |  ~energy_low]
  (junction 25) -> ACS_HOLD [order 4] : [desired_acs == uint8(3)]
  (junction 25) -> ACS_DESAT [order 8] : [desired_acs == uint8(7)]
  ACS_OPTICAL -> (junction 25) [order 1] : [desired_acs ~= uint8(8) && optical_target_available]
  (junction 25) -> ACS_OPTICAL [order 9] : [desired_acs == uint8(8)]
  (junction 25) -> ACS_SLEW_FAST [order 6] : [desired_acs == uint8(5)]
  ACS_SLEW_FAST -> (junction 25) [order 1] : [desired_acs ~= uint8(5)]
  ACS_SAFE -> (junction 25) : [desired_acs ~= uint8(9) &&...
      |  ~energy_low && recovery_ready &&...
      |  sun_sensor_valid && ~((desired_acs == uint8(2)) &&...
      |  ~reference_available) && ~((desired_acs == uint8(6)) &&...
      |  (~spin_feasible || ~spin_axis_available))]
  (junction 25) -> ACS_SAFE [order 10] : [desired_acs == uint8(9)]
  (junction 25) -> ACS_SPIN [order 7] : [desired_acs == uint8(6)]
  ACS_SPIN -> (junction 25) [order 2] : [desired_acs ~= uint8(6)]
  ACS_DESAT -> ACS_SAFE [order 2] : [energy_low]
  ACS_SLEW_FAST -> ACS_DESAT [order 3] : [wheels_saturated && ~energy_low]
  ACS_HOLD -> ACS_SAFE [order 2] : [energy_low ||...
      |  ~detumbled ||...
      |  actual_ephem == uint8(0)]
  ACS_OPTICAL -> ACS_SAFE [order 2] : [energy_low]
  ACS_SPIN -> ACS_SAFE [order 1] : [energy_low || ~spin_feasible ||...
      |  ~spin_axis_available]
  ACS_SLEW_FAST -> ACS_SAFE [order 2] : [energy_low || ~detumbled ||...
      |  actual_ephem == uint8(0)]
  data: desired_acs input uint8; actual_ephem input uint8; detumbled input boolean; reference_available input boolean; energy_low input boolean; recovery_ready input boolean; wheels_saturated input boolean; desaturated input boolean; spin_feasible input boolean; spin_axis_available input boolean; optical_target_available input boolean; sun_sensor_valid input boolean; actual_acs output uint8 =0

== stateflow chart ADCS_FSM_v1_test/Subsystem3/Mode manager/Status_Manager ==
  state STATUS
    during:
    mode_degraded = (actual_ephem ~= desired_ephem) || (actual_ads ~= desired_ads) || (actual_frame ~= desired_frame) || (actual_acs ~= desired_acs);
  (default) -> STATUS
  data: desired_ephem input uint8; desired_ads input uint8; desired_frame input uint8; desired_acs input uint8; actual_ephem input uint8; actual_ads input uint8; actual_frame input uint8; actual_acs input uint8; mode_degraded output boolean =0

== stateflow chart ADCS_FSM_v1_test/Subsystem3/Mode manager/Mode Manager/Ephemeris_Manager ==
  state EPHEM_IDLE
    entry:
    actual_ephem = uint8(0);
  state EPHEM_GPS
    entry:
    actual_ephem = uint8(2);
  state EPHEM_TLE
    entry:
    actual_ephem = uint8(1);
  EPHEM_GPS -> EPHEM_IDLE [order 1] : [desired_ephem == uint8(0)]
  EPHEM_IDLE -> EPHEM_GPS [order 2] : [desired_ephem == uint8(2)...
      |  && gps_valid]
  (default) -> EPHEM_IDLE
  EPHEM_IDLE -> EPHEM_TLE [order 1] : [desired_ephem == uint8(1) ||...
      |  (desired_ephem == uint8(2) &&...
      |  ~gps_valid && ~tle_error_high)]
  EPHEM_TLE -> EPHEM_IDLE [order 1] : [desired_ephem == uint8(0)...
      |  || tle_error_high]
  EPHEM_GPS -> EPHEM_TLE [order 2] : [desired_ephem == uint8(1) ||...
      |  ~gps_valid]
  EPHEM_TLE -> EPHEM_GPS [order 2] : [desired_ephem == uint8(2) && gps_valid]
  data: desired_ephem input uint8; gps_valid input boolean; tle_error_high input boolean; actual_ephem output uint8 =0

== stateflow chart ADCS_FSM_v1_test/Subsystem3/Mode manager/Mode Manager/ADS_Manager ==
  state ADS_IDLE
    entry:
    actual_ads = uint8(0);
  state ADS_UKF_FINE
    entry:
    actual_ads = uint8(2);
  state ADS_UKF_COARSE
    entry:
    actual_ads = uint8(1);
  ADS_UKF_FINE -> ADS_IDLE [order 2] : [desired_ads == uint8(0) || ads_fault]
  ADS_IDLE -> ADS_UKF_FINE [order 2] : [desired_ads == uint8(2) &&...
      |  ads_fine_allowed && ~ads_fault]
  (default) -> ADS_IDLE
  ADS_UKF_COARSE -> ADS_IDLE [order 1] : [desired_ads == uint8(0) || ads_fault]
  ADS_IDLE -> ADS_UKF_COARSE [order 1] : [desired_ads == uint8(1) ||...
      |  (desired_ads == uint8(2) &&...
      |  ~ads_fine_allowed)]
  ADS_UKF_FINE -> ADS_UKF_COARSE [order 1] : [desired_ads == uint8(1) ||...
      |  ~ads_fine_allowed]
  ADS_UKF_COARSE -> ADS_UKF_FINE [order 2] : [desired_ads == uint8(2) &&...
      |  ads_fine_allowed && ~ads_fault]
  data: desired_ads input uint8; ads_fine_allowed input boolean; ads_fault input boolean; actual_ads output uint8 =0

== stateflow chart ADCS_FSM_v1_test/Subsystem3/Mode manager/Mode Manager/Mission_Mode_Manager ==
  state M_DETUMBLE
    entry:
    desired_ephem = uint8(0);
    desired_ads = uint8(1);
    desired_frame = uint8(0);
    desired_acs = uint8(1);
    %desired_actuator = uint8(3);
  state M_SAFE_SUN
    entry:
    desired_ephem = uint8(0);
    desired_ads = uint8(0);
    desired_frame = uint8(0);
    desired_acs = uint8(9);
    %desired_actuator = uint8(2);
  state M_Y_SPIN
    entry:
    desired_ephem = uint8(2);
    desired_ads = uint8(1);
    desired_frame = uint8(3);
    desired_acs = uint8(6);
    %desired_actuator = uint8(2);
  state M_IDLE
    entry:
    desired_ephem = uint8(0);
    desired_ads = uint8(0);
    desired_frame = uint8(0);
    desired_acs = uint8(0);
    %desired_actuator = uint8(0);
  state M_MINMAX_DRAG
    entry:
    desired_ephem = uint8(2);
    desired_ads = uint8(2);
    desired_frame = uint8(3);
    %desired_frame = uint8(3 + 2 * drag_use_vnb);
    desired_acs = uint8(2);
    %desired_actuator = uint8(2);
  state M_POINT_NADIR
    entry:
    desired_ephem = uint8(2);
    desired_ads = uint8(2);
    desired_frame = uint8(3);
    desired_acs = uint8(2);
    %desired_actuator = uint8(2);
  state M_SLEW_FIXED
    entry:
    desired_ephem = uint8(2);
    desired_ads = uint8(2);
    desired_frame = uint8(2);
    desired_acs = uint8(4);
    %desired_actuator = uint8(2);
  state M_SLEW_FASTEST
    entry:
    desired_ephem = uint8(2);
    desired_ads = uint8(2);
    desired_frame = uint8(2);
    desired_acs = uint8(5);
    %desired_actuator = uint8(3);
  state M_POINT_MOON
    entry:
    desired_ephem = uint8(2);
    desired_ads = uint8(2);
    desired_frame = uint8(2);
    desired_acs = uint8(2);
    %desired_actuator = uint8(2);
  state M_TDI
    entry:
    desired_ephem = uint8(2);
    desired_ads = uint8(2);
    desired_frame = uint8(6);
    desired_acs = uint8(2);
    %desired_actuator = uint8(2);
  state M_POINT_SUN
    entry:
    desired_ephem = uint8(2);
    desired_ads = uint8(2);
    desired_frame = uint8(2);
    desired_acs = uint8(3);
    %desired_actuator = uint8(2);
  state M_INTERSAT_TRACK
    entry:
    desired_ephem = uint8(2);
    desired_ads = uint8(2);
    desired_frame = uint8(2);
    desired_acs = uint8(2 + 6 * intersat_sensor_tracking);
    %desired_actuator = uint8(2);
  M_DETUMBLE -> (junction 28) : [mission_cmd ~= uint8(1)]
  (junction 28) -> M_DETUMBLE [order 2] : [mission_cmd == uint8(1)]
  M_Y_SPIN -> (junction 28) : [mission_cmd ~= uint8(3)]
  M_SAFE_SUN -> (junction 28) : [mission_cmd ~= uint8(2)]
  (junction 28) -> M_SAFE_SUN [order 3] : [mission_cmd == uint8(2)]
  M_IDLE -> (junction 28) : [mission_cmd ~= uint8(0)]
  (default) -> M_IDLE
  (junction 28) -> M_IDLE [order 1] : [mission_cmd == uint8(0)]
  (junction 28) -> M_Y_SPIN [order 4] : [mission_cmd == uint8(3)]
  (junction 28) -> M_MINMAX_DRAG [order 12] : [mission_cmd == uint8(11)]
  M_MINMAX_DRAG -> (junction 28) : [mission_cmd ~= uint8(11)]
  (junction 28) -> M_POINT_NADIR [order 5] : [mission_cmd == uint8(4)]
  M_POINT_NADIR -> (junction 28) : [mission_cmd ~= uint8(4)]
  (junction 28) -> M_SLEW_FIXED [order 8] : [mission_cmd == uint8(7)]
  M_SLEW_FASTEST -> (junction 28) : [mission_cmd ~= uint8(8)]
  (junction 28) -> M_SLEW_FASTEST [order 9] : [mission_cmd == uint8(8)]
  M_SLEW_FIXED -> (junction 28) : [mission_cmd ~= uint8(7)]
  (junction 28) -> M_POINT_MOON [order 7] : [mission_cmd == uint8(6)]
  (junction 28) -> M_POINT_SUN [order 6] : [mission_cmd == uint8(5)]
  M_POINT_MOON -> (junction 28) : [mission_cmd ~= uint8(6)]
  M_POINT_SUN -> (junction 28) : [mission_cmd ~= uint8(5)]
  (junction 28) -> M_INTERSAT_TRACK [order 10] : [mission_cmd == uint8(9)]
  (junction 28) -> M_TDI [order 11] : [mission_cmd == uint8(10)]
  M_INTERSAT_TRACK -> (junction 28) : [mission_cmd ~= uint8(9)]
  M_TDI -> (junction 28) : [mission_cmd ~= uint8(10)]
  data: mission_cmd input uint8; intersat_sensor_tracking input boolean; desired_ephem output uint8 =0; desired_ads output uint8 =0; desired_frame output uint8 =0; desired_acs output uint8 =0
